simulink model "s_c_nbe_m1k"  (R2016b)
(part 3 of 198)

      settings: AttributesFormatString=Latency = %<latency>
      mask Display:
      | port_label('input', 1, 'd');
      | port_label('output', 1, 'q');
      | disp(['Z^-', num2str(latency)]);
  pipeline70 : Subsystem  AncestorBlock=casper_library_delays/pipeline  mask(pipeline){latency=2}
      mask help:
      | An explicitly laid-out delay line to avoid mapping to SRL16s
      | for use in pipelining to help achieve timing closure.
      mask init:
      | pipeline_init(gcb,'latency',latency);
      settings: AttributesFormatString=Latency = %<latency>
      mask Display:
      | port_label('input', 1, 'd');
      | port_label('output', 1, 'q');
      | disp(['Z^-', num2str(latency)]);
  pipeline71 : Subsystem  AncestorBlock=casper_library_delays/pipeline  mask(pipeline){latency=2}
      mask help:
      | An explicitly laid-out delay line to avoid mapping to SRL16s
      | for use in pipelining to help achieve timing closure.
      mask init:
      | pipeline_init(gcb,'latency',latency);
      settings: AttributesFormatString=Latency = %<latency>
      mask Display:
      | port_label('input', 1, 'd');
      | port_label('output', 1, 'q');
      | disp(['Z^-', num2str(latency)]);
  pipeline72 : Subsystem  AncestorBlock=casper_library_delays/pipeline  mask(pipeline){latency=2}
      mask help:
      | An explicitly laid-out delay line to avoid mapping to SRL16s
      | for use in pipelining to help achieve timing closure.
      mask init:
      | pipeline_init(gcb,'latency',latency);
      settings: AttributesFormatString=Latency = %<latency>
      mask Display:
      | port_label('input', 1, 'd');
      | port_label('output', 1, 'q');
      | disp(['Z^-', num2str(latency)]);
  pipeline73 : Subsystem  AncestorBlock=casper_library_delays/pipeline  mask(pipeline){latency=2}
      mask help:
      | An explicitly laid-out delay line to avoid mapping to SRL16s
      | for use in pipelining to help achieve timing closure.
      mask init:
      | pipeline_init(gcb,'latency',latency);
      settings: AttributesFormatString=Latency = %<latency>
      mask Display:
      | port_label('input', 1, 'd');
      | port_label('output', 1, 'q');
      | disp(['Z^-', num2str(latency)]);
  pipeline74 : Subsystem  AncestorBlock=casper_library_delays/pipeline  mask(pipeline){latency=2}
      mask help:
      | An explicitly laid-out delay line to avoid mapping to SRL16s
      | for use in pipelining to help achieve timing closure.
      mask init:
      | pipeline_init(gcb,'latency',latency);
      settings: AttributesFormatString=Latency = %<latency>
      mask Display:
      | port_label('input', 1, 'd');
      | port_label('output', 1, 'q');
      | disp(['Z^-', num2str(latency)]);
  pipeline75 : Subsystem  AncestorBlock=casper_library_delays/pipeline  mask(pipeline){latency=2}
      mask help:
      | An explicitly laid-out delay line to avoid mapping to SRL16s
      | for use in pipelining to help achieve timing closure.
      mask init:
      | pipeline_init(gcb,'latency',latency);
      settings: AttributesFormatString=Latency = %<latency>
      mask Display:
      | port_label('input', 1, 'd');
      | port_label('output', 1, 'q');
      | disp(['Z^-', num2str(latency)]);
  pipeline76 : Subsystem  AncestorBlock=casper_library_delays/pipeline  mask(pipeline){latency=2}
      mask help:
      | An explicitly laid-out delay line to avoid mapping to SRL16s
      | for use in pipelining to help achieve timing closure.
      mask init:
      | pipeline_init(gcb,'latency',latency);
      settings: AttributesFormatString=Latency = %<latency>
      mask Display:
      | port_label('input', 1, 'd');
      | port_label('output', 1, 'q');
      | disp(['Z^-', num2str(latency)]);
  pipeline77 : Subsystem  AncestorBlock=casper_library_delays/pipeline  mask(pipeline){latency=2}
      mask help:
      | An explicitly laid-out delay line to avoid mapping to SRL16s
      | for use in pipelining to help achieve timing closure.
      mask init:
      | pipeline_init(gcb,'latency',latency);
      settings: AttributesFormatString=Latency = %<latency>
      mask Display:
      | port_label('input', 1, 'd');
      | port_label('output', 1, 'q');
      | disp(['Z^-', num2str(latency)]);
  pipeline78 : Subsystem  AncestorBlock=casper_library_delays/pipeline  mask(pipeline){latency=2}
      mask help:
      | An explicitly laid-out delay line to avoid mapping to SRL16s
      | for use in pipelining to help achieve timing closure.
      mask init:
      | pipeline_init(gcb,'latency',latency);
      settings: AttributesFormatString=Latency = %<latency>
      mask Display:
      | port_label('input', 1, 'd');
      | port_label('output', 1, 'q');
      | disp(['Z^-', num2str(latency)]);
  pipeline79 : Subsystem  AncestorBlock=casper_library_delays/pipeline  mask(pipeline){latency=2}
      mask help:
      | An explicitly laid-out delay line to avoid mapping to SRL16s
      | for use in pipelining to help achieve timing closure.
      mask init:
      | pipeline_init(gcb,'latency',latency);
      settings: AttributesFormatString=Latency = %<latency>
      mask Display:
      | port_label('input', 1, 'd');
      | port_label('output', 1, 'q');
      | disp(['Z^-', num2str(latency)]);
  pipeline8 : Subsystem  AncestorBlock=casper_library_delays/pipeline  mask(pipeline){latency=2}
      mask help:
      | An explicitly laid-out delay line to avoid mapping to SRL16s
      | for use in pipelining to help achieve timing closure.
      mask init:
      | pipeline_init(gcb,'latency',latency);
      settings: AttributesFormatString=Latency = %<latency>
      mask Display:
      | port_label('input', 1, 'd');
      | port_label('output', 1, 'q');
      | disp(['Z^-', num2str(latency)]);
  pipeline80 : Subsystem  AncestorBlock=casper_library_delays/pipeline  mask(pipeline){latency=2}
      mask help:
      | An explicitly laid-out delay line to avoid mapping to SRL16s
      | for use in pipelining to help achieve timing closure.
      mask init:
      | pipeline_init(gcb,'latency',latency);
      settings: AttributesFormatString=Latency = %<latency>
      mask Display:
      | port_label('input', 1, 'd');
      | port_label('output', 1, 'q');
      | disp(['Z^-', num2str(latency)]);
  pipeline82 : Subsystem  AncestorBlock=casper_library_delays/pipeline  mask(pipeline){latency=2}
      mask help:
      | An explicitly laid-out delay line to avoid mapping to SRL16s
      | for use in pipelining to help achieve timing closure.
      mask init:
      | pipeline_init(gcb,'latency',latency);
      settings: AttributesFormatString=Latency = %<latency>
      mask Display:
      | port_label('input', 1, 'd');
      | port_label('output', 1, 'q');
      | disp(['Z^-', num2str(latency)]);
  pipeline83 : Subsystem  AncestorBlock=casper_library_delays/pipeline  mask(pipeline){latency=2}
      mask help:
      | An explicitly laid-out delay line to avoid mapping to SRL16s
      | for use in pipelining to help achieve timing closure.
      mask init:
      | pipeline_init(gcb,'latency',latency);
      settings: AttributesFormatString=Latency = %<latency>
      mask Display:
      | port_label('input', 1, 'd');
      | port_label('output', 1, 'q');
      | disp(['Z^-', num2str(latency)]);
  pipeline84 : Subsystem  AncestorBlock=casper_library_delays/pipeline  mask(pipeline){latency=2}
      mask help:
      | An explicitly laid-out delay line to avoid mapping to SRL16s
      | for use in pipelining to help achieve timing closure.
      mask init:
      | pipeline_init(gcb,'latency',latency);
      settings: AttributesFormatString=Latency = %<latency>
      mask Display:
      | port_label('input', 1, 'd');
      | port_label('output', 1, 'q');
      | disp(['Z^-', num2str(latency)]);
  pipeline85 : Subsystem  AncestorBlock=casper_library_delays/pipeline  mask(pipeline){latency=2}
      mask help:
      | An explicitly laid-out delay line to avoid mapping to SRL16s
      | for use in pipelining to help achieve timing closure.
      mask init:
      | pipeline_init(gcb,'latency',latency);
      settings: AttributesFormatString=Latency = %<latency>
      mask Display:
      | port_label('input', 1, 'd');
      | port_label('output', 1, 'q');
      | disp(['Z^-', num2str(latency)]);
  pipeline86 : Subsystem  AncestorBlock=casper_library_delays/pipeline  mask(pipeline){latency=2}
      mask help:
      | An explicitly laid-out delay line to avoid mapping to SRL16s
      | for use in pipelining to help achieve timing closure.
      mask init:
      | pipeline_init(gcb,'latency',latency);
      settings: AttributesFormatString=Latency = %<latency>
      mask Display:
      | port_label('input', 1, 'd');
      | port_label('output', 1, 'q');
      | disp(['Z^-', num2str(latency)]);
  pipeline87 : Subsystem  AncestorBlock=casper_library_delays/pipeline  mask(pipeline){latency=2}
      mask help:
      | An explicitly laid-out delay line to avoid mapping to SRL16s
      | for use in pipelining to help achieve timing closure.
      mask init:
      | pipeline_init(gcb,'latency',latency);
      settings: AttributesFormatString=Latency = %<latency>
      mask Display:
      | port_label('input', 1, 'd');
      | port_label('output', 1, 'q');
      | disp(['Z^-', num2str(latency)]);
  pipeline88 : Subsystem  AncestorBlock=casper_library_delays/pipeline  mask(pipeline){latency=2}
      mask help:
      | An explicitly laid-out delay line to avoid mapping to SRL16s
      | for use in pipelining to help achieve timing closure.
      mask init:
      | pipeline_init(gcb,'latency',latency);
      settings: AttributesFormatString=Latency = %<latency>
      mask Display:
      | port_label('input', 1, 'd');
      | port_label('output', 1, 'q');
      | disp(['Z^-', num2str(latency)]);
  pipeline89 : Subsystem  AncestorBlock=casper_library_delays/pipeline  mask(pipeline){latency=2}
      mask help:
      | An explicitly laid-out delay line to avoid mapping to SRL16s
      | for use in pipelining to help achieve timing closure.
      mask init:
      | pipeline_init(gcb,'latency',latency);
      settings: AttributesFormatString=Latency = %<latency>
      mask Display:
      | port_label('input', 1, 'd');
      | port_label('output', 1, 'q');
      | disp(['Z^-', num2str(latency)]);
  pipeline9 : Subsystem  AncestorBlock=casper_library_delays/pipeline  mask(pipeline){latency=2}
      mask help:
      | An explicitly laid-out delay line to avoid mapping to SRL16s
      | for use in pipelining to help achieve timing closure.
      mask init:
      | pipeline_init(gcb,'latency',latency);
      settings: AttributesFormatString=Latency = %<latency>
      mask Display:
      | port_label('input', 1, 'd');
      | port_label('output', 1, 'q');
      | disp(['Z^-', num2str(latency)]);
  pipeline90 : Subsystem  AncestorBlock=casper_library_delays/pipeline  mask(pipeline){latency=2}
      mask help:
      | An explicitly laid-out delay line to avoid mapping to SRL16s
      | for use in pipelining to help achieve timing closure.
      mask init:
      | pipeline_init(gcb,'latency',latency);
      settings: AttributesFormatString=Latency = %<latency>
      mask Display:
      | port_label('input', 1, 'd');
      | port_label('output', 1, 'q');
      | disp(['Z^-', num2str(latency)]);
  pipeline91 : Subsystem  AncestorBlock=casper_library_delays/pipeline  mask(pipeline){latency=2}
      mask help:
      | An explicitly laid-out delay line to avoid mapping to SRL16s
      | for use in pipelining to help achieve timing closure.
      mask init:
      | pipeline_init(gcb,'latency',latency);
      settings: AttributesFormatString=Latency = %<latency>
      mask Display:
      | port_label('input', 1, 'd');
      | port_label('output', 1, 'q');
      | disp(['Z^-', num2str(latency)]);
  pipeline92 : Subsystem  AncestorBlock=casper_library_delays/pipeline  mask(pipeline){latency=2}
      mask help:
      | An explicitly laid-out delay line to avoid mapping to SRL16s
      | for use in pipelining to help achieve timing closure.
      mask init:
      | pipeline_init(gcb,'latency',latency);
      settings: AttributesFormatString=Latency = %<latency>
      mask Display:
      | port_label('input', 1, 'd');
      | port_label('output', 1, 'q');
      | disp(['Z^-', num2str(latency)]);
  pipeline93 : Subsystem  AncestorBlock=casper_library_delays/pipeline  mask(pipeline){latency=2}
      mask help:
      | An explicitly laid-out delay line to avoid mapping to SRL16s
      | for use in pipelining to help achieve timing closure.
      mask init:
      | pipeline_init(gcb,'latency',latency);
      settings: AttributesFormatString=Latency = %<latency>
      mask Display:
      | port_label('input', 1, 'd');
      | port_label('output', 1, 'q');
      | disp(['Z^-', num2str(latency)]);
  pipeline94 : Subsystem  AncestorBlock=casper_library_delays/pipeline  mask(pipeline){latency=2}
      mask help:
      | An explicitly laid-out delay line to avoid mapping to SRL16s
      | for use in pipelining to help achieve timing closure.
      mask init:
      | pipeline_init(gcb,'latency',latency);
      settings: AttributesFormatString=Latency = %<latency>
      mask Display:
      | port_label('input', 1, 'd');
      | port_label('output', 1, 'q');
      | disp(['Z^-', num2str(latency)]);
  pipeline95 : Subsystem  AncestorBlock=casper_library_delays/pipeline  mask(pipeline){latency=2}
      mask help:
      | An explicitly laid-out delay line to avoid mapping to SRL16s
      | for use in pipelining to help achieve timing closure.
      mask init:
      | pipeline_init(gcb,'latency',latency);
      settings: AttributesFormatString=Latency = %<latency>
      mask Display:
      | port_label('input', 1, 'd');
      | port_label('output', 1, 'q');
      | disp(['Z^-', num2str(latency)]);
  pipeline96 : Subsystem  AncestorBlock=casper_library_delays/pipeline  mask(pipeline){latency=2}
      mask help:
      | An explicitly laid-out delay line to avoid mapping to SRL16s
      | for use in pipelining to help achieve timing closure.
      mask init:
      | pipeline_init(gcb,'latency',latency);
      settings: AttributesFormatString=Latency = %<latency>
      mask Display:
      | port_label('input', 1, 'd');
      | port_label('output', 1, 'q');
      | disp(['Z^-', num2str(latency)]);
  pipeline97 : Subsystem  AncestorBlock=casper_library_delays/pipeline  mask(pipeline){latency=2}
      mask help:
      | An explicitly laid-out delay line to avoid mapping to SRL16s
      | for use in pipelining to help achieve timing closure.
      mask init:
      | pipeline_init(gcb,'latency',latency);
      settings: AttributesFormatString=Latency = %<latency>
      mask Display:
      | port_label('input', 1, 'd');
      | port_label('output', 1, 'q');
      | disp(['Z^-', num2str(latency)]);
  pipeline98 : Subsystem  AncestorBlock=casper_library_delays/pipeline  mask(pipeline){latency=2}
      mask help:
      | An explicitly laid-out delay line to avoid mapping to SRL16s
      | for use in pipelining to help achieve timing closure.
      mask init:
      | pipeline_init(gcb,'latency',latency);
      settings: AttributesFormatString=Latency = %<latency>
      mask Display:
      | port_label('input', 1, 'd');
      | port_label('output', 1, 'q');
      | disp(['Z^-', num2str(latency)]);
  pipeline99 : Subsystem  AncestorBlock=casper_library_delays/pipeline  mask(pipeline){latency=2}
      mask help:
      | An explicitly laid-out delay line to avoid mapping to SRL16s
      | for use in pipelining to help achieve timing closure.
      mask init:
      | pipeline_init(gcb,'latency',latency);
      settings: AttributesFormatString=Latency = %<latency>
      mask Display:
      | port_label('input', 1, 'd');
      | port_label('output', 1, 'q');
      | disp(['Z^-', num2str(latency)]);
  pktlen_check : Subsystem  mask{block_len=32}
      mask prompts: block_len "Expected length"
      mask Display:
      | disp(sprintf('block_len == %i?', block_len));
      | color('green');
      | port_label('input', 1, 'pktstart')
      | port_label('input', 2, 'dv')
      | color('red');
      | port_label('output', 1, 'err')
  posedge_delay : Subsystem
  posedge_delay1 : Subsystem
  quant0 : Subsystem  mask{channel_bits=fft_stages-1, din_bit_width=18, din_bin_pt=17, coeff_bit_width=16, coeff_bin_pt=5, dout_bit_width=8, dout_bin_pt=7, overflow=Saturate, quantization=Round  (unbiased: +/- Inf), conv_latency=7, add_latency=7, mult_latency=7, bram_latency=7}
      mask prompts: channel_bits "Number channels (2^?)"; din_bit_width "Data input bit width"; din_bin_pt "Data input binary point"; coeff_bit_width "Coefficient bit width"; coeff_bin_pt "Coefficient binary point"; dout_bit_width "Data out bit width"; dout_bin_pt "Data out binary point"; overflow "Overflow behaviour"; quantization "Quantization Behaviour"; conv_latency "Conversion latency"; add_latency "Adder latency"; mult_latency "Multiplier latency"; bram_latency "BRAM latency"
      mask TypeOptions overflow: Wrap | Saturate | Error
      mask TypeOptions quantization: Truncate | Round  (unbiased: +/- Inf) | Round  (unbiased: even values)
  quant1 : Subsystem  mask{channel_bits=fft_stages-1, din_bit_width=18, din_bin_pt=17, coeff_bit_width=16, coeff_bin_pt=5, dout_bit_width=8, dout_bin_pt=7, overflow=Saturate, quantization=Round  (unbiased: +/- Inf), conv_latency=7, add_latency=7, mult_latency=7, bram_latency=7}
      mask prompts: channel_bits "Number channels (2^?)"; din_bit_width "Data input bit width"; din_bin_pt "Data input binary point"; coeff_bit_width "Coefficient bit width"; coeff_bin_pt "Coefficient binary point"; dout_bit_width "Data out bit width"; dout_bin_pt "Data out binary point"; overflow "Overflow behaviour"; quantization "Quantization Behaviour"; conv_latency "Conversion latency"; add_latency "Adder latency"; mult_latency "Multiplier latency"; bram_latency "BRAM latency"
      mask TypeOptions overflow: Wrap | Saturate | Error
      mask TypeOptions quantization: Truncate | Round  (unbiased: +/- Inf) | Round  (unbiased: even values)
  quant_pwr0 : Subsystem  Tag=xps:sw_reg  AncestorBlock=xps_library/software_register  mask(swreg){io_dir=To Processor, io_delay=0, sample_period=1, names=reg, bitwidths=32, bin_pts=31, arith_types=0, sim_port=off, show_format=off}
      mask prompts: io_dir "I/O direction"; io_delay "I/O delay"; sample_period "Sample period"; names "Bitfield names [msb...lsb]"; bitwidths "Bitfield widths"; bin_pts "Bitfield binary pts"; arith_types "Bitfield types, ufix=0, fix=1, bool=2"; sim_port "Provide sim input/output?"; show_format "Print format string?"
      mask help: A 32-bit software-accessible register. Can be divided into bitfields of varying widths and types using the fields in the block mask.
      mask init:
      | swreg_init(gcb)
      settings: AttributesFormatString=1output
      mask TypeOptions io_dir: To Processor | From Processor
      mask Callback io_dir:
      | mask_enables = get_param(gcb, 'MaskEnables');
      | mask_names = get_param(gcb, 'MaskNames');
      | if strcmp(get_param(gcb, 'io_dir'), 'To Processor'),
      |     mask_enables{ismember(mask_names, 'sample_period')} = 'off';
      | else
      |     mask_enables{ismember(mask_names, 'sample_period')} = 'on';
      | end
      | set_param(gcb, 'MaskEnables', mask_enables);
  quant_pwr1 : Subsystem  Tag=xps:sw_reg  AncestorBlock=xps_library/software_register  mask(swreg){io_dir=To Processor, io_delay=0, sample_period=1, names=reg, bitwidths=32, bin_pts=31, arith_types=0, sim_port=off, show_format=off}
      mask prompts: io_dir "I/O direction"; io_delay "I/O delay"; sample_period "Sample period"; names "Bitfield names [msb...lsb]"; bitwidths "Bitfield widths"; bin_pts "Bitfield binary pts"; arith_types "Bitfield types, ufix=0, fix=1, bool=2"; sim_port "Provide sim input/output?"; show_format "Print format string?"
      mask help: A 32-bit software-accessible register. Can be divided into bitfields of varying widths and types using the fields in the block mask.
      mask init:
      | swreg_init(gcb)
      settings: AttributesFormatString=1output
      mask TypeOptions io_dir: To Processor | From Processor
      mask Callback io_dir:
      | mask_enables = get_param(gcb, 'MaskEnables');
      | mask_names = get_param(gcb, 'MaskNames');
      | if strcmp(get_param(gcb, 'io_dir'), 'To Processor'),
      |     mask_enables{ismember(mask_names, 'sample_period')} = 'off';
      | else
      |     mask_enables{ismember(mask_names, 'sample_period')} = 'on';
      | end
      | set_param(gcb, 'MaskEnables', mask_enables);
  quant_snap_ctrl : Subsystem  Tag=xps:sw_reg  AncestorBlock=xps_library/software_register  mask(swreg){io_dir=From Processor, io_delay=0, sample_period=1, names=[single_channel channel_select], bitwidths=[1 31], bin_pts=[0 0], arith_types=[2 0], sim_port=on, show_format=on}
      mask prompts: io_dir "I/O direction"; io_delay "I/O delay"; sample_period "Sample period"; names "Bitfield names [msb...lsb]"; bitwidths "Bitfield widths"; bin_pts "Bitfield binary pts"; arith_types "Bitfield types, ufix=0, fix=1, bool=2"; sim_port "Provide sim input/output?"; show_format "Print format string?"
      mask help: A 32-bit software-accessible register. Can be divided into bitfields of varying widths and types using the fields in the block mask.
      mask init:
      | swreg_init(gcb)
      settings: AttributesFormatString=2 inputs:b,uf31.0 = 32 bits
      mask TypeOptions io_dir: To Processor | From Processor
      mask Callback io_dir:
      | mask_enables = get_param(gcb, 'MaskEnables');
      | mask_names = get_param(gcb, 'MaskNames');
      | if strcmp(get_param(gcb, 'io_dir'), 'To Processor'),
      |     mask_enables{ismember(mask_names, 'sample_period')} = 'off';
      | else
      |     mask_enables{ismember(mask_names, 'sample_period')} = 'on';
      | end
      | set_param(gcb, 'MaskEnables', mask_enables);
  quant_snap_filter0 : Subsystem
  quant_snap_filter1 : Subsystem  Commented=on
  quant_status : Subsystem  Tag=xps:sw_reg  AncestorBlock=xps_library/software register  mask(swreg){io_dir=To Processor, io_delay=0, sample_period=1, names=[pol0_or_cnt pol1_or_cnt], bitwidths=[6], bin_pts=0, arith_types=0, sim_port=off, show_format=on}
      mask prompts: io_dir "I/O direction"; io_delay "I/O delay"; sample_period "Sample period"; names "Bitfield names [msb...lsb]"; bitwidths "Bitfield widths"; bin_pts "Bitfield binary pts"; arith_types "Bitfield types, ufix=0, fix=1, bool=2"; sim_port "Provide sim input/output?"; show_format "Print format string?"
      mask help: A 32-bit software-accessible register. Can be divided into bitfields of varying widths and types using the fields in the block mask.
      mask init:
      | swreg_init(gcb)
      settings: AttributesFormatString=2 outputs:uf6.0,uf6.0 = 12 bits
      mask TypeOptions io_dir: To Processor | From Processor
      mask Callback io_dir:
      | mask_enables = get_param(gcb, 'MaskEnables');
      | mask_names = get_param(gcb, 'MaskNames');
      | if strcmp(get_param(gcb, 'io_dir'), 'To Processor'),
      |     mask_enables{ismember(mask_names, 'sample_period')} = 'off';
      | else
      |     mask_enables{ismember(mask_names, 'sample_period')} = 'on';
      | end
      | set_param(gcb, 'MaskEnables', mask_enables);
  quant_sync_cnt : Subsystem  Tag=xps:sw_reg  AncestorBlock=xps_library/Memory/software_register  mask(swreg){io_dir=To Processor, io_delay=0, init_val=0, sample_period=1, names=reg, bitwidths=8, bin_pts=0, arith_types=0, sim_port=off, show_format=on}
      mask prompts: io_dir "I/O direction"; io_delay "I/O delay"; init_val "Initial Value"; sample_period "Sample period"; names "Bitfield names [msb...lsb]"; bitwidths "Bitfield widths"; bin_pts "Bitfield binary pts"; arith_types "Bitfield types, ufix=0, fix=1, bool=2"; sim_port "Provide sim input/output?"; show_format "Print format string?"
      mask help: A 32-bit software-accessible register. Can be divided into bitfields of varying widths and types using the fields in the block mask.
      mask init:
      | swreg_init(gcb)
      settings: AttributesFormatString=1output:uf8.0 = 8 bits
      mask TypeOptions io_dir: To Processor | From Processor
      mask Callback io_dir:
      | mask_enables = get_param(gcb, 'MaskEnables');
      | mask_names = get_param(gcb, 'MaskNames');
      | if strcmp(get_param(gcb, 'io_dir'), 'To Processor'),
      |     mask_enables{ismember(mask_names, 'sample_period')} = 'off';
      | else
      |     mask_enables{ismember(mask_names, 'sample_period')} = 'on';
      | end
      | set_param(gcb, 'MaskEnables', mask_enables);
      mask DialogControl ParameterTabVar0 Prompt: Setup
  re_im_interleave : Subsystem
  reorder_status : Subsystem  Tag=xps:sw_reg  AncestorBlock=xps_library/software_register  mask(swreg){io_dir=To Processor, io_delay=0, sample_period=1, names=[timestep_err_cnt receive_err_cnt discard_cnt relock_err_cnt overflow_err_cnt dv_cnt], bitwidths=5, bin_pts=0, arith_types=0, sim_port=off, show_format=on}
      mask prompts: io_dir "I/O direction"; io_delay "I/O delay"; sample_period "Sample period"; names "Bitfield names [msb...lsb]"; bitwidths "Bitfield widths"; bin_pts "Bitfield binary pts"; arith_types "Bitfield types, ufix=0, fix=1, bool=2"; sim_port "Provide sim input/output?"; show_format "Print format string?"
      mask help: A 32-bit software-accessible register. Can be divided into bitfields of varying widths and types using the fields in the block mask.
      mask init:
      | swreg_init(gcb)
      settings: AttributesFormatString=6 outputs:uf5.0,uf5.0,uf5.0,uf5.0,uf5.0,uf5.0 = 30 bits
      mask TypeOptions io_dir: To Processor | From Processor
      mask Callback io_dir:
      | mask_enables = get_param(gcb, 'MaskEnables');
      | mask_names = get_param(gcb, 'MaskNames');
      | if strcmp(get_param(gcb, 'io_dir'), 'To Processor'),
      |     mask_enables{ismember(mask_names, 'sample_period')} = 'off';
      | else
      |     mask_enables{ismember(mask_names, 'sample_period')} = 'on';
      | end
      | set_param(gcb, 'MaskEnables', mask_enables);
  reorder_status1 : Subsystem  Tag=xps:sw_reg  AncestorBlock=xps_library/software_register  mask(swreg){io_dir=To Processor, io_delay=0, sample_period=1, names=dv_per_sec, bitwidths=32, bin_pts=0, arith_types=0, sim_port=off, show_format=on}
      mask prompts: io_dir "I/O direction"; io_delay "I/O delay"; sample_period "Sample period"; names "Bitfield names [msb...lsb]"; bitwidths "Bitfield widths"; bin_pts "Bitfield binary pts"; arith_types "Bitfield types, ufix=0, fix=1, bool=2"; sim_port "Provide sim input/output?"; show_format "Print format string?"
      mask help: A 32-bit software-accessible register. Can be divided into bitfields of varying widths and types using the fields in the block mask.
      mask init:
      | swreg_init(gcb)
      settings: AttributesFormatString=1output:uf32.0 = 32 bits
      mask TypeOptions io_dir: To Processor | From Processor
      mask Callback io_dir:
      | mask_enables = get_param(gcb, 'MaskEnables');
      | mask_names = get_param(gcb, 'MaskNames');
      | if strcmp(get_param(gcb, 'io_dir'), 'To Processor'),
      |     mask_enables{ismember(mask_names, 'sample_period')} = 'off';
      | else
      |     mask_enables{ismember(mask_names, 'sample_period')} = 'on';
      | end
      | set_param(gcb, 'MaskEnables', mask_enables);
  rx_dest_ip : Subsystem  Tag=xps:sw_reg  AncestorBlock=xps_library/software register  mask(swreg){io_dir=To Processor, io_delay=0, sample_period=1, names=reg, bitwidths=32, bin_pts=0, arith_types=0, sim_port=off, show_format=on}
      mask prompts: io_dir "I/O direction"; io_delay "I/O delay"; sample_period "Sample period"; names "Bitfield names [msb...lsb]"; bitwidths "Bitfield widths"; bin_pts "Bitfield binary pts"; arith_types "Bitfield types, ufix=0, fix=1, bool=2"; sim_port "Provide sim input/output?"; show_format "Print format string?"
      mask help: A 32-bit software-accessible register. Can be divided into bitfields of varying widths and types using the fields in the block mask.
      mask init:
      | swreg_init(gcb)
      settings: AttributesFormatString=1output:uf32.0 = 32 bits
      mask TypeOptions io_dir: To Processor | From Processor
      mask Callback io_dir:
      | mask_enables = get_param(gcb, 'MaskEnables');
      | mask_names = get_param(gcb, 'MaskNames');
      | if strcmp(get_param(gcb, 'io_dir'), 'To Processor'),
      |     mask_enables{ismember(mask_names, 'sample_period')} = 'off';
      | else
      |     mask_enables{ismember(mask_names, 'sample_period')} = 'on';
      | end
      | set_param(gcb, 'MaskEnables', mask_enables);
  snap_adc : Subsystem  Tag=casper:bitsnap  AncestorBlock=casper_library_scopes/bitfield_snapshot  mask(bitsnap){io_names=[p0_d0 p0_d1 p0_d2 p0_d3 p0_d4 p0_d5 p0_d6 p0_d7 dv sync trig trig_time], io_widths=[10 10 10 10 10 10 10 10 1 1 1 45], io_bps=[9 9 9 9 9 9 9 9 0 0 0 0], io_types=[1 1 1 1 1 1 1 1 2 2 2 0], show_format=on, snap_storage=bram, snap_dram_dimm=2, snap_dram_clock=250, snap_nsamples=8, snap_data_width=128, snap_offset=off, snap_circap=off, snap_value=off, snap_ext_arm=off, snap_ext_circ=off, snap_provide_outputs=on, snap_use_dsp48=on, snap_delay=2, extra_names=timestamp, extra_widths=32, extra_bps=0, extra_types=0}
      mask prompts: io_names "Names [msb...lsb]"; io_widths "Bitwidths [msb...lsb]"; io_bps "Binary pts [msb...lsb]"; io_types "Data types [msb...lsb], ufix=0, fix=1, bool=2"; show_format "Print format string?"; snap_storage "Storage medium"; snap_dram_dimm "DRAM dimm"; snap_dram_clock "DRAM clock rate"; snap_nsamples "Number of Samples (2^?)"; snap_data_width "Data width"; snap_offset "Start delay support"; snap_circap "Circular capture support"; snap_value "Extra value capture support"; snap_ext_arm "External arm support"; snap_ext_circ "External circular capture support"; snap_provide_outputs "Provide outputs"; snap_use_dsp48 "Use DSP48s to implement counters"; snap_delay "Pre-snapshot delay"; extra_names "Names [msb...lsb]"; extra_widths "Widths [msb...lsb]"; extra_bps "Binary pts [msb...lsb]"; extra_types "Data types [msb...lsb], ufix=0, fix=1, bool=2"
      mask help:
      | A wrapped snapshot block. Allows specification of inputs to a snapblock word so the toolflow can automatically set up the scope.
      | See documentation for snapshot for explanation of parameters.
      mask init:
      | bitsnap_init(gcb);
      settings: AttributesFormatString=|
      | snap(12):f10.9,f10.9,f10.9,f10.9,f10.9,f10.9,f10.9,f10.9,b,b,b,uf45.0 = 128 bits\n128 wide, 256 deep
      | debugID: 41370868
      mask TypeOptions snap_storage: bram | dram
      mask Callback snap_storage: bitsnap_callback();
      mask TypeOptions snap_dram_dimm: 1 | 2 | 3 | 4
      mask TypeOptions snap_dram_clock: 200 | 250 | 266 | 300 | 333
      mask TypeOptions snap_data_width: 8 | 16 | 32 | 64 | 128
      mask Callback snap_value: bitsnap_callback();
      mask Callback snap_ext_arm: bitsnap_callback();
      mask Callback snap_ext_circ: bitsnap_callback();
      mask Callback snap_provide_outputs: bitsnap_callback();
  snap_adc0 : Subsystem  Tag=casper:bitsnap  Commented=on  AncestorBlock=casper_library_scopes/bitfield_snapshot  mask(bitsnap){io_names=[p0_d0 p0_d1 p0_d2 p0_d3 p0_d4 p0_d5 p0_d6 p0_d7 dv sync], io_widths=[10 10 10 10 10 10 10 10 1 1], io_bps=[9 9 9 9 9 9 9 9 0 0], io_types=[1 1 1 1 1 1 1 1 2 2], show_format=on, snap_storage=bram, snap_dram_dimm=2, snap_dram_clock=250, snap_nsamples=10, snap_data_width=128, snap_offset=off, snap_circap=on, snap_value=on, snap_ext_arm=off, snap_ext_circ=off, snap_provide_outputs=on, snap_use_dsp48=on, snap_delay=2, extra_names=timestamp, extra_widths=32, extra_bps=0, extra_types=0}
      mask prompts: io_names "Names [msb...lsb]"; io_widths "Bitwidths [msb...lsb]"; io_bps "Binary pts [msb...lsb]"; io_types "Data types [msb...lsb], ufix=0, fix=1, bool=2"; show_format "Print format string?"; snap_storage "Storage medium"; snap_dram_dimm "DRAM dimm"; snap_dram_clock "DRAM clock rate"; snap_nsamples "Number of Samples (2^?)"; snap_data_width "Data width"; snap_offset "Start delay support"; snap_circap "Circular capture support"; snap_value "Extra value capture support"; snap_ext_arm "External arm support"; snap_ext_circ "External circular capture support"; snap_provide_outputs "Provide outputs"; snap_use_dsp48 "Use DSP48s to implement counters"; snap_delay "Pre-snapshot delay"; extra_names "Names [msb...lsb]"; extra_widths "Widths [msb...lsb]"; extra_bps "Binary pts [msb...lsb]"; extra_types "Data types [msb...lsb], ufix=0, fix=1, bool=2"
      mask help:
      | A wrapped snapshot block. Allows specification of inputs to a snapblock word so the toolflow can automatically set up the scope.
      | See documentation for snapshot for explanation of parameters.
      mask init:
      | bitsnap_init(gcb);
      settings: AttributesFormatString=|
      | snap(10):f10.9,f10.9,f10.9,f10.9,f10.9,f10.9,f10.9,f10.9,b,b = 82 bits\nextra(1):uf32.0 = 32 bits\n128 wide, 1024 deep
      | debugID: 74501914
      mask TypeOptions snap_storage: bram | dram
      mask Callback snap_storage: bitsnap_callback();
      mask TypeOptions snap_dram_dimm: 1 | 2 | 3 | 4
      mask TypeOptions snap_dram_clock: 200 | 250 | 266 | 300 | 333
      mask TypeOptions snap_data_width: 8 | 16 | 32 | 64 | 128
      mask Callback snap_value: bitsnap_callback();
      mask Callback snap_ext_arm: bitsnap_callback();
      mask Callback snap_ext_circ: bitsnap_callback();
      mask Callback snap_provide_outputs: bitsnap_callback();
  snap_adc1 : Subsystem  Tag=casper:bitsnap  Commented=on  AncestorBlock=casper_library_scopes/bitfield_snapshot  mask(bitsnap){io_names=[p1_d0 p1_d1 p1_d2 p1_d3 p1_d4 p1_d5 p1_d6 p1_d7], io_widths=10, io_bps=9, io_types=1, show_format=on, snap_storage=bram, snap_dram_dimm=2, snap_dram_clock=250, snap_nsamples=10, snap_data_width=128, snap_offset=off, snap_circap=on, snap_value=on, snap_ext_arm=off, snap_ext_circ=off, snap_provide_outputs=on, snap_use_dsp48=on, snap_delay=2, extra_names=timestamp, extra_widths=32, extra_bps=0, extra_types=0}
      mask prompts: io_names "Names [msb...lsb]"; io_widths "Bitwidths [msb...lsb]"; io_bps "Binary pts [msb...lsb]"; io_types "Data types [msb...lsb], ufix=0, fix=1, bool=2"; show_format "Print format string?"; snap_storage "Storage medium"; snap_dram_dimm "DRAM dimm"; snap_dram_clock "DRAM clock rate"; snap_nsamples "Number of Samples (2^?)"; snap_data_width "Data width"; snap_offset "Start delay support"; snap_circap "Circular capture support"; snap_value "Extra value capture support"; snap_ext_arm "External arm support"; snap_ext_circ "External circular capture support"; snap_provide_outputs "Provide outputs"; snap_use_dsp48 "Use DSP48s to implement counters"; snap_delay "Pre-snapshot delay"; extra_names "Names [msb...lsb]"; extra_widths "Widths [msb...lsb]"; extra_bps "Binary pts [msb...lsb]"; extra_types "Data types [msb...lsb], ufix=0, fix=1, bool=2"
      mask help:
      | A wrapped snapshot block. Allows specification of inputs to a snapblock word so the toolflow can automatically set up the scope.
      | See documentation for snapshot for explanation of parameters.
      mask init:
      | bitsnap_init(gcb);
      settings: AttributesFormatString=|
      | snap(8):f10.9,f10.9,f10.9,f10.9,f10.9,f10.9,f10.9,f10.9 = 80 bits\nextra(1):uf32.0 = 32 bits\n128 wide, 1024 deep
      | debugID: 74531705
      mask TypeOptions snap_storage: bram | dram
      mask Callback snap_storage: bitsnap_callback();
      mask TypeOptions snap_dram_dimm: 1 | 2 | 3 | 4
      mask TypeOptions snap_dram_clock: 200 | 250 | 266 | 300 | 333
      mask TypeOptions snap_data_width: 8 | 16 | 32 | 64 | 128
      mask Callback snap_value: bitsnap_callback();
      mask Callback snap_ext_arm: bitsnap_callback();
      mask Callback snap_ext_circ: bitsnap_callback();
      mask Callback snap_provide_outputs: bitsnap_callback();
  snap_cos : Subsystem  Tag=casper:bitsnap  AncestorBlock=casper_library_scopes/bitfield_snapshot  mask(bitsnap){io_names=[p0_d0 p0_d1 p0_d2 p0_d3 p0_d4 p0_d5 p0_d6 p0_d7 dv sync trig trig_time], io_widths=[10 10 10 10 10 10 10 10 1 1 1 44], io_bps=[9 9 9 9 9 9 9 9 0 0 0 0], io_types=[1 1 1 1 1 1 1 1 2 2 2 0], show_format=on, snap_storage=bram, snap_dram_dimm=2, snap_dram_clock=250, snap_nsamples=9, snap_data_width=128, snap_offset=off, snap_circap=off, snap_value=off, snap_ext_arm=off, snap_ext_circ=off, snap_provide_outputs=on, snap_use_dsp48=on, snap_delay=2, extra_names=timestamp, extra_widths=32, extra_bps=0, extra_types=0}
      mask prompts: io_names "Names [msb...lsb]"; io_widths "Bitwidths [msb...lsb]"; io_bps "Binary pts [msb...lsb]"; io_types "Data types [msb...lsb], ufix=0, fix=1, bool=2"; show_format "Print format string?"; snap_storage "Storage medium"; snap_dram_dimm "DRAM dimm"; snap_dram_clock "DRAM clock rate"; snap_nsamples "Number of Samples (2^?)"; snap_data_width "Data width"; snap_offset "Start delay support"; snap_circap "Circular capture support"; snap_value "Extra value capture support"; snap_ext_arm "External arm support"; snap_ext_circ "External circular capture support"; snap_provide_outputs "Provide outputs"; snap_use_dsp48 "Use DSP48s to implement counters"; snap_delay "Pre-snapshot delay"; extra_names "Names [msb...lsb]"; extra_widths "Widths [msb...lsb]"; extra_bps "Binary pts [msb...lsb]"; extra_types "Data types [msb...lsb], ufix=0, fix=1, bool=2"
      mask help:
      | A wrapped snapshot block. Allows specification of inputs to a snapblock word so the toolflow can automatically set up the scope.
      | See documentation for snapshot for explanation of parameters.
      mask init:
      | bitsnap_init(gcb);
      settings: AttributesFormatString=|
      | snap(12):f10.9,f10.9,f10.9,f10.9,f10.9,f10.9,f10.9,f10.9,b,b,b,uf44.0 = 127 bits\n128 wide, 512 deep
      | debugID: 109264557
      mask TypeOptions snap_storage: bram | dram
      mask Callback snap_storage: bitsnap_callback();
      mask TypeOptions snap_dram_dimm: 1 | 2 | 3 | 4
      mask TypeOptions snap_dram_clock: 200 | 250 | 266 | 300 | 333
      mask TypeOptions snap_data_width: 8 | 16 | 32 | 64 | 128
      mask Callback snap_value: bitsnap_callback();
      mask Callback snap_ext_arm: bitsnap_callback();
      mask Callback snap_ext_circ: bitsnap_callback();
      mask Callback snap_provide_outputs: bitsnap_callback();
  snap_dds_tg : Subsystem  Tag=casper:bitsnap  AncestorBlock=casper_library_scopes/bitfield_snapshot  mask(bitsnap){io_names=[time_slice sync dv], io_widths=[28 1 1], io_bps=[0 0 0], io_types=[0 2 2], show_format=on, snap_storage=bram, snap_dram_dimm=2, snap_dram_clock=250, snap_nsamples=9, snap_data_width=32, snap_offset=off, snap_circap=off, snap_value=off, snap_ext_arm=off, snap_ext_circ=off, snap_provide_outputs=on, snap_use_dsp48=on, snap_delay=2, extra_names=timestamp, extra_widths=32, extra_bps=0, extra_types=0}
      mask prompts: io_names "Names [msb...lsb]"; io_widths "Bitwidths [msb...lsb]"; io_bps "Binary pts [msb...lsb]"; io_types "Data types [msb...lsb], ufix=0, fix=1, bool=2"; show_format "Print format string?"; snap_storage "Storage medium"; snap_dram_dimm "DRAM dimm"; snap_dram_clock "DRAM clock rate"; snap_nsamples "Number of Samples (2^?)"; snap_data_width "Data width"; snap_offset "Start delay support"; snap_circap "Circular capture support"; snap_value "Extra value capture support"; snap_ext_arm "External arm support"; snap_ext_circ "External circular capture support"; snap_provide_outputs "Provide outputs"; snap_use_dsp48 "Use DSP48s to implement counters"; snap_delay "Pre-snapshot delay"; extra_names "Names [msb...lsb]"; extra_widths "Widths [msb...lsb]"; extra_bps "Binary pts [msb...lsb]"; extra_types "Data types [msb...lsb], ufix=0, fix=1, bool=2"
      mask help:
      | A wrapped snapshot block. Allows specification of inputs to a snapblock word so the toolflow can automatically set up the scope.
      | See documentation for snapshot for explanation of parameters.
      mask init:
      | bitsnap_init(gcb);
      settings: AttributesFormatString=|
      | snap(3):uf28.0,b,b = 30 bits\n32 wide, 512 deep
      | debugID: 44312395
      mask TypeOptions snap_storage: bram | dram
      mask Callback snap_storage: bitsnap_callback();
      mask TypeOptions snap_dram_dimm: 1 | 2 | 3 | 4
      mask TypeOptions snap_dram_clock: 200 | 250 | 266 | 300 | 333
      mask TypeOptions snap_data_width: 8 | 16 | 32 | 64 | 128
      mask Callback snap_value: bitsnap_callback();
      mask Callback snap_ext_arm: bitsnap_callback();
      mask Callback snap_ext_circ: bitsnap_callback();
      mask Callback snap_provide_outputs: bitsnap_callback();
  snap_pfbin : Subsystem  Tag=casper:bitsnap  AncestorBlock=casper_library_scopes/bitfield_snapshot  mask(bitsnap){io_names=[p0_d0 p0_d1 p0_d2 p0_d3 p0_d4 p0_d5 p0_d6 p0_d7 dv sync trig trig_time], io_widths=[10 10 10 10 10 10 10 10 1 1 1 45], io_bps=[9 9 9 9 9 9 9 9 0 0 0 0], io_types=[1 1 1 1 1 1 1 1 2 2 2 0], show_format=on, snap_storage=bram, snap_dram_dimm=2, snap_dram_clock=250, snap_nsamples=9, snap_data_width=128, snap_offset=off, snap_circap=off, snap_value=off, snap_ext_arm=off, snap_ext_circ=off, snap_provide_outputs=on, snap_use_dsp48=on, snap_delay=2, extra_names=timestamp, extra_widths=32, extra_bps=0, extra_types=0}
      mask prompts: io_names "Names [msb...lsb]"; io_widths "Bitwidths [msb...lsb]"; io_bps "Binary pts [msb...lsb]"; io_types "Data types [msb...lsb], ufix=0, fix=1, bool=2"; show_format "Print format string?"; snap_storage "Storage medium"; snap_dram_dimm "DRAM dimm"; snap_dram_clock "DRAM clock rate"; snap_nsamples "Number of Samples (2^?)"; snap_data_width "Data width"; snap_offset "Start delay support"; snap_circap "Circular capture support"; snap_value "Extra value capture support"; snap_ext_arm "External arm support"; snap_ext_circ "External circular capture support"; snap_provide_outputs "Provide outputs"; snap_use_dsp48 "Use DSP48s to implement counters"; snap_delay "Pre-snapshot delay"; extra_names "Names [msb...lsb]"; extra_widths "Widths [msb...lsb]"; extra_bps "Binary pts [msb...lsb]"; extra_types "Data types [msb...lsb], ufix=0, fix=1, bool=2"
      mask help:
      | A wrapped snapshot block. Allows specification of inputs to a snapblock word so the toolflow can automatically set up the scope.
      | See documentation for snapshot for explanation of parameters.
      mask init:
      | bitsnap_init(gcb);
      settings: AttributesFormatString=|
      | snap(12):f10.9,f10.9,f10.9,f10.9,f10.9,f10.9,f10.9,f10.9,b,b,b,uf45.0 = 128 bits\n128 wide, 512 deep
      | debugID: 53556067
      mask TypeOptions snap_storage: bram | dram
      mask Callback snap_storage: bitsnap_callback();
      mask TypeOptions snap_dram_dimm: 1 | 2 | 3 | 4
      mask TypeOptions snap_dram_clock: 200 | 250 | 266 | 300 | 333
      mask TypeOptions snap_data_width: 8 | 16 | 32 | 64 | 128
      mask Callback snap_value: bitsnap_callback();
      mask Callback snap_ext_arm: bitsnap_callback();
      mask Callback snap_ext_circ: bitsnap_callback();
      mask Callback snap_provide_outputs: bitsnap_callback();
  snap_quant0 : Subsystem  Tag=casper:bitsnap  AncestorBlock=casper_library_scopes/bitfield_snapshot  mask(bitsnap){io_names=[real0 imag0 real1 imag1 real2 imag2 real3 imag3 trig trig_time], io_widths=[8 8 8 8 8 8 8 8 1 48], io_bps=[7 7 7 7 7 7 7 7 0 0], io_types=[1 1 1 1 1 1 1 1 2 0], show_format=on, snap_storage=bram, snap_dram_dimm=2, snap_dram_clock=250, snap_nsamples=9, snap_data_width=128, snap_offset=on, snap_circap=off, snap_value=off, snap_ext_arm=off, snap_ext_circ=off, snap_provide_outputs=on, snap_use_dsp48=on, snap_delay=0, extra_names=[c d], extra_widths=[30 2], extra_bps=[0 0], extra_types=0}
      mask prompts: io_names "Names [msb...lsb]"; io_widths "Bitwidths [msb...lsb]"; io_bps "Binary pts [msb...lsb]"; io_types "Data types [msb...lsb], ufix=0, fix=1, bool=2"; show_format "Print format string?"; snap_storage "Storage medium"; snap_dram_dimm "DRAM dimm"; snap_dram_clock "DRAM clock rate"; snap_nsamples "Number of Samples (2^?)"; snap_data_width "Data width"; snap_offset "Start delay support"; snap_circap "Circular capture support"; snap_value "Extra value capture support"; snap_ext_arm "External arm support"; snap_ext_circ "External circular capture support"; snap_provide_outputs "Provide outputs"; snap_use_dsp48 "Use DSP48s to implement counters"; snap_delay "Pre-snapshot delay"; extra_names "Names [msb...lsb]"; extra_widths "Widths [msb...lsb]"; extra_bps "Binary pts [msb...lsb]"; extra_types "Data types [msb...lsb], ufix=0, fix=1, bool=2"
      mask help:
      | A wrapped snapshot block. Allows specification of inputs to a snapblock word so the toolflow can automatically set up the scope.
      | See documentation for snapshot for explanation of parameters.
      mask init:
      | bitsnap_init(gcb);
      settings: AttributesFormatString=|
      | snap(10):f8.7,f8.7,f8.7,f8.7,f8.7,f8.7,f8.7,f8.7,b,uf48.0 = 113 bits\n128 wide, 512 deep
      | debugID: 23153533
      mask TypeOptions snap_storage: bram | dram
      mask Callback snap_storage: bitsnap_callback();
      mask TypeOptions snap_dram_dimm: 1 | 2 | 3 | 4
      mask TypeOptions snap_dram_clock: 200 | 250 | 266 | 300 | 333
      mask TypeOptions snap_data_width: 8 | 16 | 32 | 64 | 128
      mask Callback snap_value: bitsnap_callback();
      mask Callback snap_ext_arm: bitsnap_callback();
      mask Callback snap_ext_circ: bitsnap_callback();
      mask Callback snap_provide_outputs: bitsnap_callback();
  snap_quant1 : Subsystem  Tag=casper:bitsnap  Commented=on  AncestorBlock=casper_library_scopes/bitfield_snapshot  mask(bitsnap){io_names=[real0 imag0 real1 imag1 real2 imag2 real3 imag3], io_widths=8, io_bps=7, io_types=1, show_format=on, snap_storage=bram, snap_dram_dimm=2, snap_dram_clock=250, snap_nsamples=10, snap_data_width=64, snap_offset=on, snap_circap=off, snap_value=off, snap_ext_arm=off, snap_ext_circ=off, snap_provide_outputs=on, snap_use_dsp48=on, snap_delay=0, extra_names=[c d], extra_widths=[30 2], extra_bps=[0 0], extra_types=0}
      mask prompts: io_names "Names [msb...lsb]"; io_widths "Bitwidths [msb...lsb]"; io_bps "Binary pts [msb...lsb]"; io_types "Data types [msb...lsb], ufix=0, fix=1, bool=2"; show_format "Print format string?"; snap_storage "Storage medium"; snap_dram_dimm "DRAM dimm"; snap_dram_clock "DRAM clock rate"; snap_nsamples "Number of Samples (2^?)"; snap_data_width "Data width"; snap_offset "Start delay support"; snap_circap "Circular capture support"; snap_value "Extra value capture support"; snap_ext_arm "External arm support"; snap_ext_circ "External circular capture support"; snap_provide_outputs "Provide outputs"; snap_use_dsp48 "Use DSP48s to implement counters"; snap_delay "Pre-snapshot delay"; extra_names "Names [msb...lsb]"; extra_widths "Widths [msb...lsb]"; extra_bps "Binary pts [msb...lsb]"; extra_types "Data types [msb...lsb], ufix=0, fix=1, bool=2"
      mask help:
      | A wrapped snapshot block. Allows specification of inputs to a snapblock word so the toolflow can automatically set up the scope.
      | See documentation for snapshot for explanation of parameters.
      mask init:
      | bitsnap_init(gcb);
      settings: AttributesFormatString=|
      | snap(8):f8.7,f8.7,f8.7,f8.7,f8.7,f8.7,f8.7,f8.7 = 64 bits\n64 wide, 1024 deep
      | debugID: 23183324
      mask TypeOptions snap_storage: bram | dram
      mask Callback snap_storage: bitsnap_callback();
      mask TypeOptions snap_dram_dimm: 1 | 2 | 3 | 4
      mask TypeOptions snap_dram_clock: 200 | 250 | 266 | 300 | 333
      mask TypeOptions snap_data_width: 8 | 16 | 32 | 64 | 128
      mask Callback snap_value: bitsnap_callback();
      mask Callback snap_ext_arm: bitsnap_callback();
      mask Callback snap_ext_circ: bitsnap_callback();
      mask Callback snap_provide_outputs: bitsnap_callback();
  snap_sync_gen : Subsystem  Tag=casper:bitsnap  AncestorBlock=casper_library_scopes/bitfield_snapshot  mask(bitsnap){io_names=[synced_delay sync_timeout pack_sync board_in_fault time synced sync_armed time_diff_err timestep_err cd_err ct_err], io_widths=[1 1 1 1 48 1 1 1 1 1 1], io_bps=0, io_types=[2 2 2 2 0 2 2 2 2 2 2], show_format=on, snap_storage=bram, snap_dram_dimm=2, snap_dram_clock=250, snap_nsamples=8, snap_data_width=64, snap_offset=off, snap_circap=on, snap_value=off, snap_ext_arm=off, snap_ext_circ=off, snap_provide_outputs=on, snap_use_dsp48=on, snap_delay=2, extra_names=timestamp, extra_widths=32, extra_bps=0, extra_types=0}
      mask prompts: io_names "Names [msb...lsb]"; io_widths "Bitwidths [msb...lsb]"; io_bps "Binary pts [msb...lsb]"; io_types "Data types [msb...lsb], ufix=0, fix=1, bool=2"; show_format "Print format string?"; snap_storage "Storage medium"; snap_dram_dimm "DRAM dimm"; snap_dram_clock "DRAM clock rate"; snap_nsamples "Number of Samples (2^?)"; snap_data_width "Data width"; snap_offset "Start delay support"; snap_circap "Circular capture support"; snap_value "Extra value capture support"; snap_ext_arm "External arm support"; snap_ext_circ "External circular capture support"; snap_provide_outputs "Provide outputs"; snap_use_dsp48 "Use DSP48s to implement counters"; snap_delay "Pre-snapshot delay"; extra_names "Names [msb...lsb]"; extra_widths "Widths [msb...lsb]"; extra_bps "Binary pts [msb...lsb]"; extra_types "Data types [msb...lsb], ufix=0, fix=1, bool=2"
      mask help:
      | A wrapped snapshot block. Allows specification of inputs to a snapblock word so the toolflow can automatically set up the scope.
      | See documentation for snapshot for explanation of parameters.
      mask init:
      | bitsnap_init(gcb);
      settings: AttributesFormatString=|
      | snap(11):b,b,b,b,uf48.0,b,b,b,b,b,b = 58 bits\n64 wide, 256 deep
      | debugID: 65383422
      mask TypeOptions snap_storage: bram | dram
      mask Callback snap_storage: bitsnap_callback();
      mask TypeOptions snap_dram_dimm: 1 | 2 | 3 | 4
      mask TypeOptions snap_dram_clock: 200 | 250 | 266 | 300 | 333
      mask TypeOptions snap_data_width: 8 | 16 | 32 | 64 | 128
      mask Callback snap_value: bitsnap_callback();
      mask Callback snap_ext_arm: bitsnap_callback();
      mask Callback snap_ext_circ: bitsnap_callback();
      mask Callback snap_provide_outputs: bitsnap_callback();
  snap_time_check : Subsystem  Tag=casper:bitsnap  Commented=on  AncestorBlock=casper_library_scopes/bitfield_snapshot  mask(bitsnap){io_names=[time80_48 pack_sync_time time_diff], io_widths=[48 48 32], io_bps=0, io_types=[0 0 1], show_format=on, snap_storage=bram, snap_dram_dimm=2, snap_dram_clock=250, snap_nsamples=8, snap_data_width=128, snap_offset=off, snap_circap=off, snap_value=off, snap_ext_arm=off, snap_ext_circ=off, snap_provide_outputs=on, snap_use_dsp48=on, snap_delay=2, extra_names=timestamp, extra_widths=32, extra_bps=0, extra_types=0}
      mask prompts: io_names "Names [msb...lsb]"; io_widths "Bitwidths [msb...lsb]"; io_bps "Binary pts [msb...lsb]"; io_types "Data types [msb...lsb], ufix=0, fix=1, bool=2"; show_format "Print format string?"; snap_storage "Storage medium"; snap_dram_dimm "DRAM dimm"; snap_dram_clock "DRAM clock rate"; snap_nsamples "Number of Samples (2^?)"; snap_data_width "Data width"; snap_offset "Start delay support"; snap_circap "Circular capture support"; snap_value "Extra value capture support"; snap_ext_arm "External arm support"; snap_ext_circ "External circular capture support"; snap_provide_outputs "Provide outputs"; snap_use_dsp48 "Use DSP48s to implement counters"; snap_delay "Pre-snapshot delay"; extra_names "Names [msb...lsb]"; extra_widths "Widths [msb...lsb]"; extra_bps "Binary pts [msb...lsb]"; extra_types "Data types [msb...lsb], ufix=0, fix=1, bool=2"
      mask help:
      | A wrapped snapshot block. Allows specification of inputs to a snapblock word so the toolflow can automatically set up the scope.
      | See documentation for snapshot for explanation of parameters.
      mask init:
      | bitsnap_init(gcb);
      settings: AttributesFormatString=|
      | snap(3):uf48.0,uf48.0,f32.0 = 128 bits\n128 wide, 256 deep
      | debugID: 49026964
      mask TypeOptions snap_storage: bram | dram
      mask Callback snap_storage: bitsnap_callback();
      mask TypeOptions snap_dram_dimm: 1 | 2 | 3 | 4
      mask TypeOptions snap_dram_clock: 200 | 250 | 266 | 300 | 333
      mask TypeOptions snap_data_width: 8 | 16 | 32 | 64 | 128
      mask Callback snap_value: bitsnap_callback();
      mask Callback snap_ext_arm: bitsnap_callback();
      mask Callback snap_ext_circ: bitsnap_callback();
      mask Callback snap_provide_outputs: bitsnap_callback();
  ss_time_trig_adc : Subsystem
  ss_time_trig_pfbin : Subsystem
  ss_time_trig_pfbin1 : Subsystem
  ss_time_trig_quant : Subsystem
  ss_trig_time_in_lsw : Subsystem  Tag=xps:sw_reg  AncestorBlock=xps_library/Memory/software_register  mask(swreg){io_dir=From Processor, io_delay=1, init_val=0, sample_period=1, names=time, bitwidths=32, bin_pts=0, arith_types=0, sim_port=on, show_format=on}
      mask prompts: io_dir "I/O direction"; io_delay "I/O delay"; init_val "Initial Value"; sample_period "Sample period"; names "Bitfield names [msb...lsb]"; bitwidths "Bitfield widths"; bin_pts "Bitfield binary pts"; arith_types "Bitfield types, ufix=0, fix=1, bool=2"; sim_port "Provide sim input/output?"; show_format "Print format string?"
      mask help: A 32-bit software-accessible register. Can be divided into bitfields of varying widths and types using the fields in the block mask.
      mask init:
      | swreg_init(gcb)
      settings: AttributesFormatString=1input:uf32.0 = 32 bits
      mask TypeOptions io_dir: To Processor | From Processor
      mask Callback io_dir:
      | mask_enables = get_param(gcb, 'MaskEnables');
      | mask_names = get_param(gcb, 'MaskNames');
      | if strcmp(get_param(gcb, 'io_dir'), 'To Processor'),
      |     mask_enables{ismember(mask_names, 'sample_period')} = 'off';
      | else
      |     mask_enables{ismember(mask_names, 'sample_period')} = 'on';
      | end
      | set_param(gcb, 'MaskEnables', mask_enables);
      mask DialogControl ParameterTabVar0 Prompt: Setup
  ss_trig_time_in_msw : Subsystem  Tag=xps:sw_reg  AncestorBlock=xps_library/Memory/software_register  mask(swreg){io_dir=From Processor, io_delay=1, init_val=0, sample_period=1, names=time, bitwidths=16, bin_pts=0, arith_types=0, sim_port=on, show_format=on}
      mask prompts: io_dir "I/O direction"; io_delay "I/O delay"; init_val "Initial Value"; sample_period "Sample period"; names "Bitfield names [msb...lsb]"; bitwidths "Bitfield widths"; bin_pts "Bitfield binary pts"; arith_types "Bitfield types, ufix=0, fix=1, bool=2"; sim_port "Provide sim input/output?"; show_format "Print format string?"
      mask help: A 32-bit software-accessible register. Can be divided into bitfields of varying widths and types using the fields in the block mask.
      mask init:
      | swreg_init(gcb)
      settings: AttributesFormatString=1input:uf16.0 = 16 bits
      mask TypeOptions io_dir: To Processor | From Processor
      mask Callback io_dir:
      | mask_enables = get_param(gcb, 'MaskEnables');
      | mask_names = get_param(gcb, 'MaskNames');
      | if strcmp(get_param(gcb, 'io_dir'), 'To Processor'),
      |     mask_enables{ismember(mask_names, 'sample_period')} = 'off';
      | else
      |     mask_enables{ismember(mask_names, 'sample_period')} = 'on';
      | end
      | set_param(gcb, 'MaskEnables', mask_enables);
      mask DialogControl ParameterTabVar0 Prompt: Setup
  sync_gen : Subsystem  mask{zerolsbs=26}
      mask prompts: zerolsbs "No. LSBs to be zero:"
  sync_mangle : Subsystem
  sync_status0 : Subsystem  Tag=xps:sw_reg  AncestorBlock=xps_library/software_register  mask(swreg){io_dir=To Processor, io_delay=0, sample_period=1, names=[synced_delay board_in_fault synced sync_armed sync_ct sync_flag sync_pack], bitwidths=[1 1 1 1 8 8 8], bin_pts=0, arith_types=[2 2 2 2 0 0 0], sim_port=off, show_format=on}
      mask prompts: io_dir "I/O direction"; io_delay "I/O delay"; sample_period "Sample period"; names "Bitfield names [msb...lsb]"; bitwidths "Bitfield widths"; bin_pts "Bitfield binary pts"; arith_types "Bitfield types, ufix=0, fix=1, bool=2"; sim_port "Provide sim input/output?"; show_format "Print format string?"
      mask help: A 32-bit software-accessible register. Can be divided into bitfields of varying widths and types using the fields in the block mask.
      mask init:
      | swreg_init(gcb)
      settings: AttributesFormatString=7 outputs:b,b,b,b,uf8.0,uf8.0,uf8.0 = 28 bits
      mask TypeOptions io_dir: To Processor | From Processor
      mask Callback io_dir:
      | mask_enables = get_param(gcb, 'MaskEnables');
      | mask_names = get_param(gcb, 'MaskNames');
      | if strcmp(get_param(gcb, 'io_dir'), 'To Processor'),
      |     mask_enables{ismember(mask_names, 'sample_period')} = 'off';
      | else
      |     mask_enables{ismember(mask_names, 'sample_period')} = 'on';
      | end
      | set_param(gcb, 'MaskEnables', mask_enables);
  sync_status1 : Subsystem  Tag=xps:sw_reg  AncestorBlock=xps_library/software register  mask(swreg){io_dir=To Processor, io_delay=0, sample_period=1, names=[timeout_resync_cnt time_diff_resync_cnt timestep_resync_cnt cd_resync_cnt ct_resync_cnt fault_clear_timeout_cnt fault_present_timeout_cnt], bitwidths=4, bin_pts=0, arith_types=0, sim_port=off, show_format=on}
      mask prompts: io_dir "I/O direction"; io_delay "I/O delay"; sample_period "Sample period"; names "Bitfield names [msb...lsb]"; bitwidths "Bitfield widths"; bin_pts "Bitfield binary pts"; arith_types "Bitfield types, ufix=0, fix=1, bool=2"; sim_port "Provide sim input/output?"; show_format "Print format string?"
      mask help: A 32-bit software-accessible register. Can be divided into bitfields of varying widths and types using the fields in the block mask.
      mask init:
      | swreg_init(gcb)
      settings: AttributesFormatString=7 outputs:uf4.0,uf4.0,uf4.0,uf4.0,uf4.0,uf4.0,uf4.0 = 28 bits
      mask TypeOptions io_dir: To Processor | From Processor
      mask Callback io_dir:
      | mask_enables = get_param(gcb, 'MaskEnables');
      | mask_names = get_param(gcb, 'MaskNames');
      | if strcmp(get_param(gcb, 'io_dir'), 'To Processor'),
      |     mask_enables{ismember(mask_names, 'sample_period')} = 'off';
      | else
      |     mask_enables{ismember(mask_names, 'sample_period')} = 'on';
      | end
      | set_param(gcb, 'MaskEnables', mask_enables);
  sync_status2 : Subsystem  Tag=xps:sw_reg  AncestorBlock=xps_library/software_register  mask(swreg){io_dir=To Processor, io_delay=0, sample_period=1, names=[sync80_cnt sync_pfb_cnt sync_fdfs_cnt sync_quant_cnt], bitwidths=8, bin_pts=0, arith_types=0, sim_port=off, show_format=on}
      mask prompts: io_dir "I/O direction"; io_delay "I/O delay"; sample_period "Sample period"; names "Bitfield names [msb...lsb]"; bitwidths "Bitfield widths"; bin_pts "Bitfield binary pts"; arith_types "Bitfield types, ufix=0, fix=1, bool=2"; sim_port "Provide sim input/output?"; show_format "Print format string?"
      mask help: A 32-bit software-accessible register. Can be divided into bitfields of varying widths and types using the fields in the block mask.
      mask init:
      | swreg_init(gcb)
      settings: AttributesFormatString=4 outputs:uf8.0,uf8.0,uf8.0,uf8.0 = 32 bits
      mask TypeOptions io_dir: To Processor | From Processor
      mask Callback io_dir:
      | mask_enables = get_param(gcb, 'MaskEnables');
      | mask_names = get_param(gcb, 'MaskNames');
      | if strcmp(get_param(gcb, 'io_dir'), 'To Processor'),
      |     mask_enables{ismember(mask_names, 'sample_period')} = 'off';
      | else
      |     mask_enables{ismember(mask_names, 'sample_period')} = 'on';
      | end
      | set_param(gcb, 'MaskEnables', mask_enables);
  sync_time_lsw : Subsystem  Tag=xps:sw_reg  AncestorBlock=xps_library/software_register  mask(swreg){io_dir=To Processor, io_delay=0, sample_period=1, names=reg, bitwidths=32, bin_pts=0, arith_types=0, sim_port=off, show_format=on}
      mask prompts: io_dir "I/O direction"; io_delay "I/O delay"; sample_period "Sample period"; names "Bitfield names [msb...lsb]"; bitwidths "Bitfield widths"; bin_pts "Bitfield binary pts"; arith_types "Bitfield types, ufix=0, fix=1, bool=2"; sim_port "Provide sim input/output?"; show_format "Print format string?"
      mask help: A 32-bit software-accessible register. Can be divided into bitfields of varying widths and types using the fields in the block mask.
      mask init:
      | swreg_init(gcb)
      settings: AttributesFormatString=1output:uf32.0 = 32 bits
      mask TypeOptions io_dir: To Processor | From Processor
      mask Callback io_dir:
      | mask_enables = get_param(gcb, 'MaskEnables');
      | mask_names = get_param(gcb, 'MaskNames');
      | if strcmp(get_param(gcb, 'io_dir'), 'To Processor'),
      |     mask_enables{ismember(mask_names, 'sample_period')} = 'off';
      | else
      |     mask_enables{ismember(mask_names, 'sample_period')} = 'on';
      | end
      | set_param(gcb, 'MaskEnables', mask_enables);
  sync_time_msw : Subsystem  Tag=xps:sw_reg  AncestorBlock=xps_library/software_register  mask(swreg){io_dir=To Processor, io_delay=0, sample_period=1, names=reg, bitwidths=16, bin_pts=0, arith_types=0, sim_port=off, show_format=on}
      mask prompts: io_dir "I/O direction"; io_delay "I/O delay"; sample_period "Sample period"; names "Bitfield names [msb...lsb]"; bitwidths "Bitfield widths"; bin_pts "Bitfield binary pts"; arith_types "Bitfield types, ufix=0, fix=1, bool=2"; sim_port "Provide sim input/output?"; show_format "Print format string?"
      mask help: A 32-bit software-accessible register. Can be divided into bitfields of varying widths and types using the fields in the block mask.
      mask init:
      | swreg_init(gcb)
      settings: AttributesFormatString=1output:uf16.0 = 16 bits
      mask TypeOptions io_dir: To Processor | From Processor
      mask Callback io_dir:
      | mask_enables = get_param(gcb, 'MaskEnables');
      | mask_names = get_param(gcb, 'MaskNames');
      | if strcmp(get_param(gcb, 'io_dir'), 'To Processor'),
      |     mask_enables{ismember(mask_names, 'sample_period')} = 'off';
      | else
      |     mask_enables{ismember(mask_names, 'sample_period')} = 'on';
      | end
      | set_param(gcb, 'MaskEnables', mask_enables);
  time_check : Subsystem  Tag=xps:sw_reg  AncestorBlock=xps_library/software register  mask(swreg){io_dir=From Processor, io_delay=0, sample_period=1, names=[max_difference], bitwidths=[32], bin_pts=[0], arith_types=[0], sim_port=off, show_format=on}
      mask prompts: io_dir "I/O direction"; io_delay "I/O delay"; sample_period "Sample period"; names "Bitfield names [msb...lsb]"; bitwidths "Bitfield widths"; bin_pts "Bitfield binary pts"; arith_types "Bitfield types, ufix=0, fix=1, bool=2"; sim_port "Provide sim input/output?"; show_format "Print format string?"
      mask help: A 32-bit software-accessible register. Can be divided into bitfields of varying widths and types using the fields in the block mask.
      mask init:
      | swreg_init(gcb)
      settings: AttributesFormatString=1input:uf32.0 = 32 bits
      mask TypeOptions io_dir: To Processor | From Processor
      mask Callback io_dir:
      | mask_enables = get_param(gcb, 'MaskEnables');
      | mask_names = get_param(gcb, 'MaskNames');
      | if strcmp(get_param(gcb, 'io_dir'), 'To Processor'),
      |     mask_enables{ismember(mask_names, 'sample_period')} = 'off';
      | else
      |     mask_enables{ismember(mask_names, 'sample_period')} = 'on';
      | end
      | set_param(gcb, 'MaskEnables', mask_enables);
  time_difference : Subsystem  Tag=xps:sw_reg  AncestorBlock=xps_library/software register  mask(swreg){io_dir=To Processor, io_delay=0, sample_period=1, names=time_difference, bitwidths=32, bin_pts=0, arith_types=1, sim_port=off, show_format=on}
      mask prompts: io_dir "I/O direction"; io_delay "I/O delay"; sample_period "Sample period"; names "Bitfield names [msb...lsb]"; bitwidths "Bitfield widths"; bin_pts "Bitfield binary pts"; arith_types "Bitfield types, ufix=0, fix=1, bool=2"; sim_port "Provide sim input/output?"; show_format "Print format string?"
      mask help: A 32-bit software-accessible register. Can be divided into bitfields of varying widths and types using the fields in the block mask.
      mask init:
      | swreg_init(gcb)
      settings: AttributesFormatString=1output:f32.0 = 32 bits
      mask TypeOptions io_dir: To Processor | From Processor
      mask Callback io_dir:
      | mask_enables = get_param(gcb, 'MaskEnables');
      | mask_names = get_param(gcb, 'MaskNames');
      | if strcmp(get_param(gcb, 'io_dir'), 'To Processor'),
      |     mask_enables{ismember(mask_names, 'sample_period')} = 'off';
      | else
      |     mask_enables{ismember(mask_names, 'sample_period')} = 'on';
      | end
      | set_param(gcb, 'MaskEnables', mask_enables);
  time_gen : Subsystem  mask{n_bits_period=fft_stages-1-2, n_bits_increment=3, n_bits_counter=48-fft_stages}
      mask prompts: n_bits_period "Period (2^?)"; n_bits_increment "Increment (2^?)"; n_bits_counter "Counter size (2^?)"
  time_gen1 : Subsystem  mask{n_bits_period=fft_stages-1-2-1+8, n_bits_increment=3, n_bits_counter=48-(fft_stages+8)}
      mask prompts: n_bits_period "Period (2^?)"; n_bits_increment "Increment (2^?)"; n_bits_counter "Counter size (2^?)"
  time_gen_cd : Subsystem  mask{n_bits_period=fft_stages-1-2, n_bits_increment=0, n_bits_counter=48-fft_stages}
      mask prompts: n_bits_period "Period (2^?)"; n_bits_increment "Increment (2^?)"; n_bits_counter "Counter size (2^?)"
  time_gen_dds : Subsystem  mask{n_bits_period=0, n_bits_increment=3, n_bits_counter=48}
      mask prompts: n_bits_period "Period (2^?)"; n_bits_increment "Increment (2^?)"; n_bits_counter "Counter size (2^?)"
  tl_cd0 : Subsystem  mask(timed_latch){n_bits_time=48-fft_stages, n_bits_quantization=fft_stages, n_bits_counters=4}
      mask prompts: n_bits_time "Number bits in time to compare"; n_bits_quantization "Time offset from lsb"; n_bits_counters "Bits in status counters"
      mask help:
      | Latches load_value when armed and current_time matches requested time.
      | current_time should be in ADC samples.
      mask init:
      | set_param([gcb,'/status'], 'bitwidths', mat2str([1, repmat(n_bits_counters, 1, 2)]));
      mask Help:
      | When armed, will latch new value when current time matches the time
      | specified. The input time should be in samples and mask settings allow
      | a portion of this to be compared to cater for quantization. Arm and latch
      | counts allow the current state, pending and missed latch events to be
      | determined.
  tl_cd0_control : Subsystem  Tag=xps:sw_reg  AncestorBlock=xps_library/software_register  mask(swreg){io_dir=From Processor, io_delay=0, sample_period=1, names=load_time_lsw, bitwidths=32, bin_pts=0, arith_types=0, sim_port=on, show_format=on}
      mask prompts: io_dir "I/O direction"; io_delay "I/O delay"; sample_period "Sample period"; names "Bitfield names [msb...lsb]"; bitwidths "Bitfield widths"; bin_pts "Bitfield binary pts"; arith_types "Bitfield types, ufix=0, fix=1, bool=2"; sim_port "Provide sim input/output?"; show_format "Print format string?"
      mask help: A 32-bit software-accessible register. Can be divided into bitfields of varying widths and types using the fields in the block mask.
      mask init:
      | swreg_init(gcb)
      settings: AttributesFormatString=1input:uf32.0 = 32 bits
      mask TypeOptions io_dir: To Processor | From Processor
      mask Callback io_dir:
      | mask_enables = get_param(gcb, 'MaskEnables');
      | mask_names = get_param(gcb, 'MaskNames');
      | if strcmp(get_param(gcb, 'io_dir'), 'To Processor'),
      |     mask_enables{ismember(mask_names, 'sample_period')} = 'off';
      | else
      |     mask_enables{ismember(mask_names, 'sample_period')} = 'on';
      | end
      | set_param(gcb, 'MaskEnables', mask_enables);
  tl_cd0_control0 : Subsystem  Tag=xps:sw_reg  AncestorBlock=xps_library/software_register  mask(swreg){io_dir=From Processor, io_delay=0, sample_period=1, names=[arm load_immediate load_time_msw], bitwidths=[1 1 16], bin_pts=[0 0 0], arith_types=[2 2 0], sim_port=on, show_format=on}
      mask prompts: io_dir "I/O direction"; io_delay "I/O delay"; sample_period "Sample period"; names "Bitfield names [msb...lsb]"; bitwidths "Bitfield widths"; bin_pts "Bitfield binary pts"; arith_types "Bitfield types, ufix=0, fix=1, bool=2"; sim_port "Provide sim input/output?"; show_format "Print format string?"
      mask help: A 32-bit software-accessible register. Can be divided into bitfields of varying widths and types using the fields in the block mask.
      mask init:
      | swreg_init(gcb)
      settings: AttributesFormatString=3 inputs:b,b,uf16.0 = 18 bits
      mask TypeOptions io_dir: To Processor | From Processor
      mask Callback io_dir:
      | mask_enables = get_param(gcb, 'MaskEnables');
      | mask_names = get_param(gcb, 'MaskNames');
      | if strcmp(get_param(gcb, 'io_dir'), 'To Processor'),
      |     mask_enables{ismember(mask_names, 'sample_period')} = 'off';
      | else
      |     mask_enables{ismember(mask_names, 'sample_period')} = 'on';
      | end
      | set_param(gcb, 'MaskEnables', mask_enables);
  tl_cd1 : Subsystem  mask(timed_latch){n_bits_time=48-fft_stages, n_bits_quantization=fft_stages, n_bits_counters=4}
      mask prompts: n_bits_time "Number bits in time to compare"; n_bits_quantization "Time offset from lsb"; n_bits_counters "Bits in status counters"
      mask help:
      | Latches load_value when armed and current_time matches requested time.
      | current_time should be in ADC samples.
      mask init:
      | set_param([gcb,'/status'], 'bitwidths', mat2str([1, repmat(n_bits_counters, 1, 2)]));
      mask Help:
      | When armed, will latch new value when current time matches the time
      | specified. The input time should be in samples and mask settings allow
      | a portion of this to be compared to cater for quantization. Arm and latch
      | counts allow the current state, pending and missed latch events to be
      | determined.
  tl_cd1_control : Subsystem  Tag=xps:sw_reg  AncestorBlock=xps_library/software_register  mask(swreg){io_dir=From Processor, io_delay=0, sample_period=1, names=load_time_lsw, bitwidths=32, bin_pts=0, arith_types=0, sim_port=on, show_format=on}
      mask prompts: io_dir "I/O direction"; io_delay "I/O delay"; sample_period "Sample period"; names "Bitfield names [msb...lsb]"; bitwidths "Bitfield widths"; bin_pts "Bitfield binary pts"; arith_types "Bitfield types, ufix=0, fix=1, bool=2"; sim_port "Provide sim input/output?"; show_format "Print format string?"
      mask help: A 32-bit software-accessible register. Can be divided into bitfields of varying widths and types using the fields in the block mask.
      mask init:
      | swreg_init(gcb)
      settings: AttributesFormatString=1input:uf32.0 = 32 bits
      mask TypeOptions io_dir: To Processor | From Processor
      mask Callback io_dir:
      | mask_enables = get_param(gcb, 'MaskEnables');
      | mask_names = get_param(gcb, 'MaskNames');
      | if strcmp(get_param(gcb, 'io_dir'), 'To Processor'),
      |     mask_enables{ismember(mask_names, 'sample_period')} = 'off';
      | else
      |     mask_enables{ismember(mask_names, 'sample_period')} = 'on';
      | end
      | set_param(gcb, 'MaskEnables', mask_enables);
  tl_cd1_control0 : Subsystem  Tag=xps:sw_reg  AncestorBlock=xps_library/software_register  mask(swreg){io_dir=From Processor, io_delay=0, sample_period=1, names=[arm load_immediate load_time_msw], bitwidths=[1 1 16], bin_pts=[0 0 0], arith_types=[2 2 0], sim_port=on, show_format=on}
      mask prompts: io_dir "I/O direction"; io_delay "I/O delay"; sample_period "Sample period"; names "Bitfield names [msb...lsb]"; bitwidths "Bitfield widths"; bin_pts "Bitfield binary pts"; arith_types "Bitfield types, ufix=0, fix=1, bool=2"; sim_port "Provide sim input/output?"; show_format "Print format string?"
      mask help: A 32-bit software-accessible register. Can be divided into bitfields of varying widths and types using the fields in the block mask.
      mask init:
      | swreg_init(gcb)
      settings: AttributesFormatString=3 inputs:b,b,uf16.0 = 18 bits
      mask TypeOptions io_dir: To Processor | From Processor
      mask Callback io_dir:
      | mask_enables = get_param(gcb, 'MaskEnables');
      | mask_names = get_param(gcb, 'MaskNames');
      | if strcmp(get_param(gcb, 'io_dir'), 'To Processor'),
      |     mask_enables{ismember(mask_names, 'sample_period')} = 'off';
      | else
      |     mask_enables{ismember(mask_names, 'sample_period')} = 'on';
      | end
      | set_param(gcb, 'MaskEnables', mask_enables);
  tl_cd_bs0 : Subsystem  mask(timed_latch){n_bits_time=48-fft_stages, n_bits_quantization=fft_stages, n_bits_counters=4}
      mask prompts: n_bits_time "Number bits in time to compare"; n_bits_quantization "Time offset from lsb"; n_bits_counters "Bits in status counters"
      mask help:
      | Latches load_value when armed and current_time matches requested time.
      | current_time should be in ADC samples.
      mask init:
      | set_param([gcb,'/status'], 'bitwidths', mat2str([1, repmat(n_bits_counters, 1, 2)]));
      mask Help:
      | When armed, will latch new value when current time matches the time
      | specified. The input time should be in samples and mask settings allow
      | a portion of this to be compared to cater for quantization. Arm and latch
      | counts allow the current state, pending and missed latch events to be
      | determined.
  tl_cd_bs1 : Subsystem  mask(timed_latch){n_bits_time=48-fft_stages, n_bits_quantization=fft_stages, n_bits_counters=4}
      mask prompts: n_bits_time "Number bits in time to compare"; n_bits_quantization "Time offset from lsb"; n_bits_counters "Bits in status counters"
      mask help:
      | Latches load_value when armed and current_time matches requested time.
      | current_time should be in ADC samples.
      mask init:
      | set_param([gcb,'/status'], 'bitwidths', mat2str([1, repmat(n_bits_counters, 1, 2)]));
      mask Help:
      | When armed, will latch new value when current time matches the time
      | specified. The input time should be in samples and mask settings allow
      | a portion of this to be compared to cater for quantization. Arm and latch
      | counts allow the current state, pending and missed latch events to be
      | determined.
  tl_fd0 : Subsystem  mask(timed_latch){n_bits_time=48-fft_stages, n_bits_quantization=fft_stages, n_bits_counters=4}
      mask prompts: n_bits_time "Number bits in time to compare"; n_bits_quantization "Time offset from lsb"; n_bits_counters "Bits in status counters"
      mask help:
      | Latches load_value when armed and current_time matches requested time.
      | current_time should be in ADC samples.
      mask init:
      | set_param([gcb,'/status'], 'bitwidths', mat2str([1, repmat(n_bits_counters, 1, 2)]));
      mask Help:
      | When armed, will latch new value when current time matches the time
      | specified. The input time should be in samples and mask settings allow
      | a portion of this to be compared to cater for quantization. Arm and latch
      | counts allow the current state, pending and missed latch events to be
      | determined.
  tl_fd1 : Subsystem  mask(timed_latch){n_bits_time=48-fft_stages, n_bits_quantization=fft_stages, n_bits_counters=4}
      mask prompts: n_bits_time "Number bits in time to compare"; n_bits_quantization "Time offset from lsb"; n_bits_counters "Bits in status counters"
      mask help:
      | Latches load_value when armed and current_time matches requested time.
      | current_time should be in ADC samples.
      mask init:
      | set_param([gcb,'/status'], 'bitwidths', mat2str([1, repmat(n_bits_counters, 1, 2)]));
      mask Help:
      | When armed, will latch new value when current time matches the time
      | specified. The input time should be in samples and mask settings allow
      | a portion of this to be compared to cater for quantization. Arm and latch
      | counts allow the current state, pending and missed latch events to be
      | determined.
  trig_level : Subsystem  Tag=xps:sw_reg  Commented=on  AncestorBlock=xps_library/software register  mask(swreg){io_dir=From Processor, io_delay=0, sample_period=1, names=level, bitwidths=10, bin_pts=9, arith_types=1, sim_port=off, show_format=on}
      mask prompts: io_dir "I/O direction"; io_delay "I/O delay"; sample_period "Sample period"; names "Bitfield names [msb...lsb]"; bitwidths "Bitfield widths"; bin_pts "Bitfield binary pts"; arith_types "Bitfield types, ufix=0, fix=1, bool=2"; sim_port "Provide sim input/output?"; show_format "Print format string?"
      mask help: A 32-bit software-accessible register. Can be divided into bitfields of varying widths and types using the fields in the block mask.
      mask init:
      | swreg_init(gcb)
      settings: AttributesFormatString=1input:f10.9 = 10 bits
      mask TypeOptions io_dir: To Processor | From Processor
      mask Callback io_dir:
      | mask_enables = get_param(gcb, 'MaskEnables');
      | mask_names = get_param(gcb, 'MaskNames');
      | if strcmp(get_param(gcb, 'io_dir'), 'To Processor'),
      |     mask_enables{ismember(mask_names, 'sample_period')} = 'off';
      | else
      |     mask_enables{ismember(mask_names, 'sample_period')} = 'on';
      | end
      | set_param(gcb, 'MaskEnables', mask_enables);
  trig_time_lsw : Subsystem  Tag=xps:sw_reg  Commented=on  AncestorBlock=xps_library/software register  mask(swreg){io_dir=From Processor, io_delay=0, sample_period=1, names=lsw, bitwidths=32, bin_pts=0, arith_types=0, sim_port=off, show_format=on}
      mask prompts: io_dir "I/O direction"; io_delay "I/O delay"; sample_period "Sample period"; names "Bitfield names [msb...lsb]"; bitwidths "Bitfield widths"; bin_pts "Bitfield binary pts"; arith_types "Bitfield types, ufix=0, fix=1, bool=2"; sim_port "Provide sim input/output?"; show_format "Print format string?"
      mask help: A 32-bit software-accessible register. Can be divided into bitfields of varying widths and types using the fields in the block mask.
      mask init:
      | swreg_init(gcb)
      settings: AttributesFormatString=1input:uf32.0 = 32 bits
      mask TypeOptions io_dir: To Processor | From Processor
      mask Callback io_dir:
      | mask_enables = get_param(gcb, 'MaskEnables');
      | mask_names = get_param(gcb, 'MaskNames');
      | if strcmp(get_param(gcb, 'io_dir'), 'To Processor'),
      |     mask_enables{ismember(mask_names, 'sample_period')} = 'off';
      | else
      |     mask_enables{ismember(mask_names, 'sample_period')} = 'on';
      | end
      | set_param(gcb, 'MaskEnables', mask_enables);
  trig_time_msw : Subsystem  Tag=xps:sw_reg  Commented=on  AncestorBlock=xps_library/software register  mask(swreg){io_dir=From Processor, io_delay=0, sample_period=1, names=msw, bitwidths=16, bin_pts=0, arith_types=0, sim_port=off, show_format=on}
      mask prompts: io_dir "I/O direction"; io_delay "I/O delay"; sample_period "Sample period"; names "Bitfield names [msb...lsb]"; bitwidths "Bitfield widths"; bin_pts "Bitfield binary pts"; arith_types "Bitfield types, ufix=0, fix=1, bool=2"; sim_port "Provide sim input/output?"; show_format "Print format string?"
      mask help: A 32-bit software-accessible register. Can be divided into bitfields of varying widths and types using the fields in the block mask.
      mask init:
      | swreg_init(gcb)
      settings: AttributesFormatString=1input:uf16.0 = 16 bits
      mask TypeOptions io_dir: To Processor | From Processor
      mask Callback io_dir:
      | mask_enables = get_param(gcb, 'MaskEnables');
      | mask_names = get_param(gcb, 'MaskNames');
      | if strcmp(get_param(gcb, 'io_dir'), 'To Processor'),
      |     mask_enables{ismember(mask_names, 'sample_period')} = 'off';
      | else
      |     mask_enables{ismember(mask_names, 'sample_period')} = 'on';
      | end
      | set_param(gcb, 'MaskEnables', mask_enables);
  ts_ss_lock : Subsystem  Tag=xps:sw_reg  AncestorBlock=xps_library/Memory/software_register  mask(swreg){io_dir=From Processor, io_delay=1, init_val=0, sample_period=1, names=en, bitwidths=1, bin_pts=0, arith_types=2, sim_port=on, show_format=on}
      mask prompts: io_dir "I/O direction"; io_delay "I/O delay"; init_val "Initial Value"; sample_period "Sample period"; names "Bitfield names [msb...lsb]"; bitwidths "Bitfield widths"; bin_pts "Bitfield binary pts"; arith_types "Bitfield types, ufix=0, fix=1, bool=2"; sim_port "Provide sim input/output?"; show_format "Print format string?"
      mask help: A 32-bit software-accessible register. Can be divided into bitfields of varying widths and types using the fields in the block mask.
      mask init:
      | swreg_init(gcb)
      settings: AttributesFormatString=1input:b = 1 bits
      mask TypeOptions io_dir: To Processor | From Processor
      mask Callback io_dir:
      | mask_enables = get_param(gcb, 'MaskEnables');
      | mask_names = get_param(gcb, 'MaskNames');
      | if strcmp(get_param(gcb, 'io_dir'), 'To Processor'),
      |     mask_enables{ismember(mask_names, 'sample_period')} = 'off';
      | else
      |     mask_enables{ismember(mask_names, 'sample_period')} = 'on';
      | end
      | set_param(gcb, 'MaskEnables', mask_enables);
      mask DialogControl ParameterTabVar0 Prompt: Setup
  ts_tvg : Subsystem
  tvg : Subsystem
  tvg_tone_levels : Subsystem  Tag=xps:sw_reg  AncestorBlock=xps_library/software_register  mask(swreg){io_dir=From Processor, io_delay=0, sample_period=1, names=[p0r p0i p1r p1i], bitwidths=8, bin_pts=7, arith_types=1, sim_port=on, show_format=on}
      mask prompts: io_dir "I/O direction"; io_delay "I/O delay"; sample_period "Sample period"; names "Bitfield names [msb...lsb]"; bitwidths "Bitfield widths"; bin_pts "Bitfield binary pts"; arith_types "Bitfield types, ufix=0, fix=1, bool=2"; sim_port "Provide sim input/output?"; show_format "Print format string?"
      mask help: A 32-bit software-accessible register. Can be divided into bitfields of varying widths and types using the fields in the block mask.
      mask init:
      | swreg_init(gcb)
      settings: AttributesFormatString=4 inputs:f8.7,f8.7,f8.7,f8.7 = 32 bits
      mask TypeOptions io_dir: To Processor | From Processor
      mask Callback io_dir:
      | mask_enables = get_param(gcb, 'MaskEnables');
      | mask_names = get_param(gcb, 'MaskNames');
      | if strcmp(get_param(gcb, 'io_dir'), 'To Processor'),
      |     mask_enables{ismember(mask_names, 'sample_period')} = 'off';
      | else
      |     mask_enables{ismember(mask_names, 'sample_period')} = 'on';
      | end
      | set_param(gcb, 'MaskEnables', mask_enables);
  tvg_tone_targets : Subsystem  Tag=xps:sw_reg  AncestorBlock=xps_library/software_register  mask(swreg){io_dir=From Processor, io_delay=0, sample_period=1, names=[p0 p1], bitwidths=fft_stages, bin_pts=0, arith_types=0, sim_port=on, show_format=on}
      mask prompts: io_dir "I/O direction"; io_delay "I/O delay"; sample_period "Sample period"; names "Bitfield names [msb...lsb]"; bitwidths "Bitfield widths"; bin_pts "Bitfield binary pts"; arith_types "Bitfield types, ufix=0, fix=1, bool=2"; sim_port "Provide sim input/output?"; show_format "Print format string?"
      mask help: A 32-bit software-accessible register. Can be divided into bitfields of varying widths and types using the fields in the block mask.
      mask init:
      | swreg_init(gcb)
      settings: AttributesFormatString=2 inputs:uf11.0,uf11.0 = 22 bits
      mask TypeOptions io_dir: To Processor | From Processor
      mask Callback io_dir:
      | mask_enables = get_param(gcb, 'MaskEnables');
      | mask_names = get_param(gcb, 'MaskNames');
      | if strcmp(get_param(gcb, 'io_dir'), 'To Processor'),
      |     mask_enables{ismember(mask_names, 'sample_period')} = 'off';
      | else
      |     mask_enables{ismember(mask_names, 'sample_period')} = 'on';
      | end
      | set_param(gcb, 'MaskEnables', mask_enables);
  tx_metadata : Subsystem  Tag=xps:sw_reg  AncestorBlock=xps_library/software register  mask(swreg){io_dir=From Processor, io_delay=0, sample_period=1, names=[porttx board_id], bitwidths=[16 8], bin_pts=0, arith_types=0, sim_port=off, show_format=on}
      mask prompts: io_dir "I/O direction"; io_delay "I/O delay"; sample_period "Sample period"; names "Bitfield names [msb...lsb]"; bitwidths "Bitfield widths"; bin_pts "Bitfield binary pts"; arith_types "Bitfield types, ufix=0, fix=1, bool=2"; sim_port "Provide sim input/output?"; show_format "Print format string?"
      mask help: A 32-bit software-accessible register. Can be divided into bitfields of varying widths and types using the fields in the block mask.
      mask init:
      | swreg_init(gcb)
      settings: AttributesFormatString=2 inputs:uf16.0,uf8.0 = 24 bits
      mask TypeOptions io_dir: To Processor | From Processor
      mask Callback io_dir:
      | mask_enables = get_param(gcb, 'MaskEnables');
      | mask_names = get_param(gcb, 'MaskNames');
      | if strcmp(get_param(gcb, 'io_dir'), 'To Processor'),
      |     mask_enables{ismember(mask_names, 'sample_period')} = 'off';
      | else
      |     mask_enables{ismember(mask_names, 'sample_period')} = 'on';
      | end
      | set_param(gcb, 'MaskEnables', mask_enables);
  unpack : Subsystem
  unpack_status : Subsystem  Tag=xps:sw_reg  AncestorBlock=xps_library/software_register  mask(swreg){io_dir=To Processor, io_delay=0, sample_period=1, names=[magic_err_cnt header_err_cnt pad_err_cnt pkt_len_err_cnt time_err_cnt], bitwidths=6, bin_pts=0, arith_types=0, sim_port=off, show_format=on}
      mask prompts: io_dir "I/O direction"; io_delay "I/O delay"; sample_period "Sample period"; names "Bitfield names [msb...lsb]"; bitwidths "Bitfield widths"; bin_pts "Bitfield binary pts"; arith_types "Bitfield types, ufix=0, fix=1, bool=2"; sim_port "Provide sim input/output?"; show_format "Print format string?"
      mask help: A 32-bit software-accessible register. Can be divided into bitfields of varying widths and types using the fields in the block mask.
      mask init:
      | swreg_init(gcb)
      settings: AttributesFormatString=5 outputs:uf6.0,uf6.0,uf6.0,uf6.0,uf6.0 = 30 bits
      mask TypeOptions io_dir: To Processor | From Processor
      mask Callback io_dir:
      | mask_enables = get_param(gcb, 'MaskEnables');
      | mask_names = get_param(gcb, 'MaskNames');
      | if strcmp(get_param(gcb, 'io_dir'), 'To Processor'),
      |     mask_enables{ismember(mask_names, 'sample_period')} = 'off';
      | else
      |     mask_enables{ismember(mask_names, 'sample_period')} = 'on';
      | end
      | set_param(gcb, 'MaskEnables', mask_enables);
  unpack_status1 : Subsystem  Tag=xps:sw_reg  AncestorBlock=xps_library/software_register  mask(swreg){io_dir=To Processor, io_delay=0, sample_period=1, names=pkt_cnt, bitwidths=32, bin_pts=0, arith_types=0, sim_port=off, show_format=on}
      mask prompts: io_dir "I/O direction"; io_delay "I/O delay"; sample_period "Sample period"; names "Bitfield names [msb...lsb]"; bitwidths "Bitfield widths"; bin_pts "Bitfield binary pts"; arith_types "Bitfield types, ufix=0, fix=1, bool=2"; sim_port "Provide sim input/output?"; show_format "Print format string?"
      mask help: A 32-bit software-accessible register. Can be divided into bitfields of varying widths and types using the fields in the block mask.
      mask init:
      | swreg_init(gcb)
      settings: AttributesFormatString=1output:uf32.0 = 32 bits
      mask TypeOptions io_dir: To Processor | From Processor
      mask Callback io_dir:
      | mask_enables = get_param(gcb, 'MaskEnables');
      | mask_names = get_param(gcb, 'MaskNames');
      | if strcmp(get_param(gcb, 'io_dir'), 'To Processor'),
      |     mask_enables{ismember(mask_names, 'sample_period')} = 'off';
      | else
      |     mask_enables{ismember(mask_names, 'sample_period')} = 'on';
      | end
      | set_param(gcb, 'MaskEnables', mask_enables);
  wb_prog_delay : Subsystem  mask{n_bits_fft=fft_stages, n_bits_cd=32}
      mask prompts: n_bits_fft "fft length (2^?)"; n_bits_cd "max coarse delay (2^?)"
  wb_prog_delay1 : Subsystem  mask{n_bits_fft=fft_stages, n_bits_cd=32}
      mask prompts: n_bits_fft "fft length (2^?)"; n_bits_cd "max coarse delay (2^?)"
  we_delay1 : Subsystem  AncestorBlock=casper_library_delays/pipeline  mask(pipeline){latency=2}
      mask help:
      | An explicitly laid-out delay line to avoid mapping to SRL16s
      | for use in pipelining to help achieve timing closure.
      mask init:
      | pipeline_init(gcb,'latency',latency);
      settings: AttributesFormatString=Latency = %<latency>
      mask Display:
      | port_label('input', 1, 'd');
      | port_label('output', 1, 'q');
      | disp(['Z^-', num2str(latency)]);
  we_delay112 : Subsystem  AncestorBlock=casper_library_delays/pipeline  mask(pipeline){latency=2}
      mask help:
      | An explicitly laid-out delay line to avoid mapping to SRL16s
      | for use in pipelining to help achieve timing closure.
      mask init:
      | pipeline_init(gcb,'latency',latency);
      settings: AttributesFormatString=Latency = %<latency>
      mask Display:
      | port_label('input', 1, 'd');
      | port_label('output', 1, 'q');
      | disp(['Z^-', num2str(latency)]);
  we_delay113 : Subsystem  AncestorBlock=casper_library_delays/pipeline  mask(pipeline){latency=2}
      mask help:
      | An explicitly laid-out delay line to avoid mapping to SRL16s
      | for use in pipelining to help achieve timing closure.
      mask init:
      | pipeline_init(gcb,'latency',latency);
      settings: AttributesFormatString=Latency = %<latency>
      mask Display:
      | port_label('input', 1, 'd');
      | port_label('output', 1, 'q');
      | disp(['Z^-', num2str(latency)]);
  we_delay114 : Subsystem  AncestorBlock=casper_library_delays/pipeline  mask(pipeline){latency=2}
      mask help:
      | An explicitly laid-out delay line to avoid mapping to SRL16s
      | for use in pipelining to help achieve timing closure.
      mask init:
      | pipeline_init(gcb,'latency',latency);
      settings: AttributesFormatString=Latency = %<latency>
      mask Display:
      | port_label('input', 1, 'd');
      | port_label('output', 1, 'q');
      | disp(['Z^-', num2str(latency)]);
  we_delay115 : Subsystem  AncestorBlock=casper_library_delays/pipeline  mask(pipeline){latency=2}
      mask help:
      | An explicitly laid-out delay line to avoid mapping to SRL16s
      | for use in pipelining to help achieve timing closure.
      mask init:
      | pipeline_init(gcb,'latency',latency);
      settings: AttributesFormatString=Latency = %<latency>
      mask Display:
      | port_label('input', 1, 'd');
      | port_label('output', 1, 'q');
      | disp(['Z^-', num2str(latency)]);
  we_delay116 : Subsystem  AncestorBlock=casper_library_delays/pipeline  mask(pipeline){latency=2}
      mask help:
      | An explicitly laid-out delay line to avoid mapping to SRL16s
      | for use in pipelining to help achieve timing closure.
      mask init:
      | pipeline_init(gcb,'latency',latency);
      settings: AttributesFormatString=Latency = %<latency>
      mask Display:
      | port_label('input', 1, 'd');
      | port_label('output', 1, 'q');
      | disp(['Z^-', num2str(latency)]);
  we_delay117 : Subsystem  AncestorBlock=casper_library_delays/pipeline  mask(pipeline){latency=2}
      mask help:
      | An explicitly laid-out delay line to avoid mapping to SRL16s
      | for use in pipelining to help achieve timing closure.
      mask init:
      | pipeline_init(gcb,'latency',latency);
      settings: AttributesFormatString=Latency = %<latency>
      mask Display:
      | port_label('input', 1, 'd');
      | port_label('output', 1, 'q');
      | disp(['Z^-', num2str(latency)]);
  we_delay124 : Subsystem  AncestorBlock=casper_library_delays/pipeline  mask(pipeline){latency=2}
      mask help:
      | An explicitly laid-out delay line to avoid mapping to SRL16s
      | for use in pipelining to help achieve timing closure.
      mask init:
      | pipeline_init(gcb,'latency',latency);
      settings: AttributesFormatString=Latency = %<latency>
      mask Display:
      | port_label('input', 1, 'd');
      | port_label('output', 1, 'q');
      | disp(['Z^-', num2str(latency)]);
  we_delay126 : Subsystem  AncestorBlock=casper_library_delays/pipeline  mask(pipeline){latency=2}
      mask help:
      | An explicitly laid-out delay line to avoid mapping to SRL16s
      | for use in pipelining to help achieve timing closure.
      mask init:
      | pipeline_init(gcb,'latency',latency);
      settings: AttributesFormatString=Latency = %<latency>
      mask Display:
      | port_label('input', 1, 'd');
      | port_label('output', 1, 'q');
      | disp(['Z^-', num2str(latency)]);
  we_delay13 : Subsystem  AncestorBlock=casper_library_delays/pipeline  mask(pipeline){latency=2}
      mask help:
      | An explicitly laid-out delay line to avoid mapping to SRL16s
      | for use in pipelining to help achieve timing closure.
      mask init:
      | pipeline_init(gcb,'latency',latency);
      settings: AttributesFormatString=Latency = %<latency>
      mask Display:
      | port_label('input', 1, 'd');
      | port_label('output', 1, 'q');
      | disp(['Z^-', num2str(latency)]);
  we_delay2 : Subsystem  AncestorBlock=casper_library_delays/pipeline  mask(pipeline){latency=2}
      mask help:
      | An explicitly laid-out delay line to avoid mapping to SRL16s
      | for use in pipelining to help achieve timing closure.
      mask init:
      | pipeline_init(gcb,'latency',latency);
      settings: AttributesFormatString=Latency = %<latency>
      mask Display:
      | port_label('input', 1, 'd');
      | port_label('output', 1, 'q');
      | disp(['Z^-', num2str(latency)]);
  we_delay29 : Subsystem  AncestorBlock=casper_library_delays/pipeline  mask(pipeline){latency=2}
      mask help:
      | An explicitly laid-out delay line to avoid mapping to SRL16s
      | for use in pipelining to help achieve timing closure.
      mask init:
      | pipeline_init(gcb,'latency',latency);
      settings: AttributesFormatString=Latency = %<latency>
      mask Display:
      | port_label('input', 1, 'd');
      | port_label('output', 1, 'q');
      | disp(['Z^-', num2str(latency)]);
  we_delay37 : Subsystem  AncestorBlock=casper_library_delays/pipeline  mask(pipeline){latency=2}
      mask help:
      | An explicitly laid-out delay line to avoid mapping to SRL16s
      | for use in pipelining to help achieve timing closure.
      mask init:
      | pipeline_init(gcb,'latency',latency);
      settings: AttributesFormatString=Latency = %<latency>
      mask Display:
      | port_label('input', 1, 'd');
      | port_label('output', 1, 'q');
      | disp(['Z^-', num2str(latency)]);
  we_delay38 : Subsystem  AncestorBlock=casper_library_delays/pipeline  mask(pipeline){latency=2}
      mask help:
      | An explicitly laid-out delay line to avoid mapping to SRL16s
      | for use in pipelining to help achieve timing closure.
      mask init:
      | pipeline_init(gcb,'latency',latency);
      settings: AttributesFormatString=Latency = %<latency>
      mask Display:
      | port_label('input', 1, 'd');
      | port_label('output', 1, 'q');
      | disp(['Z^-', num2str(latency)]);
  we_delay39 : Subsystem  AncestorBlock=casper_library_delays/pipeline  mask(pipeline){latency=2}
      mask help:
      | An explicitly laid-out delay line to avoid mapping to SRL16s
      | for use in pipelining to help achieve timing closure.
      mask init:
      | pipeline_init(gcb,'latency',latency);
      settings: AttributesFormatString=Latency = %<latency>
      mask Display:
      | port_label('input', 1, 'd');
      | port_label('output', 1, 'q');
      | disp(['Z^-', num2str(latency)]);
  we_delay41 : Subsystem  AncestorBlock=casper_library_delays/pipeline  mask(pipeline){latency=2}
      mask help:
      | An explicitly laid-out delay line to avoid mapping to SRL16s
      | for use in pipelining to help achieve timing closure.
      mask init:
      | pipeline_init(gcb,'latency',latency);
      settings: AttributesFormatString=Latency = %<latency>
      mask Display:
      | port_label('input', 1, 'd');
      | port_label('output', 1, 'q');
      | disp(['Z^-', num2str(latency)]);
  we_delay47 : Subsystem  AncestorBlock=casper_library_delays/pipeline  mask(pipeline){latency=2}
      mask help:
      | An explicitly laid-out delay line to avoid mapping to SRL16s
      | for use in pipelining to help achieve timing closure.
      mask init:
      | pipeline_init(gcb,'latency',latency);
      settings: AttributesFormatString=Latency = %<latency>
      mask Display:
      | port_label('input', 1, 'd');
      | port_label('output', 1, 'q');
      | disp(['Z^-', num2str(latency)]);
  we_delay48 : Subsystem  AncestorBlock=casper_library_delays/pipeline  mask(pipeline){latency=2}
      mask help:
      | An explicitly laid-out delay line to avoid mapping to SRL16s
      | for use in pipelining to help achieve timing closure.
      mask init:
      | pipeline_init(gcb,'latency',latency);
      settings: AttributesFormatString=Latency = %<latency>
      mask Display:
      | port_label('input', 1, 'd');
      | port_label('output', 1, 'q');
      | disp(['Z^-', num2str(latency)]);
  we_delay49 : Subsystem  AncestorBlock=casper_library_delays/pipeline  mask(pipeline){latency=2}
      mask help:
      | An explicitly laid-out delay line to avoid mapping to SRL16s
      | for use in pipelining to help achieve timing closure.
      mask init:
      | pipeline_init(gcb,'latency',latency);
      settings: AttributesFormatString=Latency = %<latency>
      mask Display:
      | port_label('input', 1, 'd');
      | port_label('output', 1, 'q');
      | disp(['Z^-', num2str(latency)]);
  we_delay50 : Subsystem  AncestorBlock=casper_library_delays/pipeline  mask(pipeline){latency=2}
      mask help:
      | An explicitly laid-out delay line to avoid mapping to SRL16s
      | for use in pipelining to help achieve timing closure.
      mask init:
      | pipeline_init(gcb,'latency',latency);
      settings: AttributesFormatString=Latency = %<latency>
      mask Display:
      | port_label('input', 1, 'd');
      | port_label('output', 1, 'q');
      | disp(['Z^-', num2str(latency)]);
  we_delay7 : Subsystem  AncestorBlock=casper_library_delays/pipeline  mask(pipeline){latency=2}
      mask help:
      | An explicitly laid-out delay line to avoid mapping to SRL16s
      | for use in pipelining to help achieve timing closure.
      mask init:
      | pipeline_init(gcb,'latency',latency);
      settings: AttributesFormatString=Latency = %<latency>
      mask Display:
      | port_label('input', 1, 'd');
      | port_label('output', 1, 'q');
      | disp(['Z^-', num2str(latency)]);
  x_setup : Subsystem  Tag=xps:sw_reg  AncestorBlock=xps_library/software_register  mask(swreg){io_dir=From Processor, io_delay=0, sample_period=1, names=[f_per_x ip_per_x num_x snap_arm pktstart_mux pack_mux pktoffset_sel], bitwidths=[15 4 9 1 1 1 1], bin_pts=[0 2 0 0 0 0 0], arith_types=[0 0 0 2 0 2 0], sim_port=off, show_format=on}
      mask prompts: io_dir "I/O direction"; io_delay "I/O delay"; sample_period "Sample period"; names "Bitfield names [msb...lsb]"; bitwidths "Bitfield widths"; bin_pts "Bitfield binary pts"; arith_types "Bitfield types, ufix=0, fix=1, bool=2"; sim_port "Provide sim input/output?"; show_format "Print format string?"
      mask help: A 32-bit software-accessible register. Can be divided into bitfields of varying widths and types using the fields in the block mask.
      mask init:
      | swreg_init(gcb)
      settings: AttributesFormatString=7 inputs:uf15.0,uf4.2,uf9.0,b,uf1.0,b,uf1.0 = 32 bits
      mask TypeOptions io_dir: To Processor | From Processor
      mask Callback io_dir:
      | mask_enables = get_param(gcb, 'MaskEnables');
      | mask_names = get_param(gcb, 'MaskNames');
      | if strcmp(get_param(gcb, 'io_dir'), 'To Processor'),
      |     mask_enables{ismember(mask_names, 'sample_period')} = 'off';
      | else
      |     mask_enables{ismember(mask_names, 'sample_period')} = 'on';
      | end
      | set_param(gcb, 'MaskEnables', mask_enables);
      mask DialogControl ParameterTabVar0 Prompt: Setup
  xsg_core_config : Subsystem  Tag=xps:xsg  AncestorBlock=xps_library/XSG_core_config  mask(xsg core config){hw_sys=SKARAB:xc7vx690t, clk_src=sys_clk, clk_rate=238, sample_period=1, synthesis_tool=XST}
      mask prompts: hw_sys "Hardware Platform"; clk_src "User IP Clock source"; clk_rate "User IP Clock Rate (MHz)"; sample_period "Sample Period"; synthesis_tool "Synthesis Tool:"
      mask help:
      | The XSG Core Config block is used to configure the System Generator design
      | for the casper_xps toolflow. Settings here are used to configure the
      | Xilinx System Generator block parameters automatically, and control toolflow
      | script  execution. It needs to be at the top level of all designs being compiled
      | with the casper_xps toolflow.
      mask init:
      | xps_xsg_conf_mask;
      mask Help: eval('xlWeb([getenv(''MLIB_ROOT''), ''\doc\html\sys_xsg_core_config\sys_xsg_core_config.html''])')
      mask TypeOptions hw_sys: ROACH:sx95t | ROACH:lx110t | ROACH2:sx475t | SNAP:xc7k160t | KC705:xc7k325t | SKARAB:xc7vx690t
      mask Callback hw_sys: xps_xsg_conf_callback
      mask TypeOptions clk_src: sys_clk | aux_clk
      mask Callback clk_src: xps_xsg_conf_callback
      mask Callback clk_rate: xps_xsg_conf_callback
      mask TypeOptions synthesis_tool: Leonardo Spectrum | Synplify | Synplify Pro | XST
      mask Display: fprintf(['MSSGE\n', hw_sys]);
  tag scope: arm_ts_ss_lock=global, arm_ts_ss_rst=global, cnt_rst=global, ct_board_hmc_offset=global, ct_chans_per_board=global, ct_chans_per_x=global, ct_chans_per_x_recip=global, ct_fake_data_error=global, ct_freq_gen_offset=global, ct_num_x_boards=global, ct_num_x_boards_recip=global, ct_num_xeng=global, ct_num_xeng_recip=global, ct_rst_err_latch=global, ct_tag_insert_sel=global, ct_tvg_en2=global, ct_tvg_en=global, ct_x_per_board=global, ct_x_per_board_recip=global, force_gbe_txen=global, local_time_capture=global, local_time_src=global, obuf_read_gap=global, pfb_bypass=global, pktoffset_sel=global, pktstart_sel=global, reo_time_change=global, snap_reord_mux_we_sel=global, snap_stop_mux_sel=global, ss_trig_time_in=global, sys_rst=global, tg_dds_time_out=global, tg_rd_time_out=global, time80_48=global, ts_ss_lock=global, ts_tvg_en=global, tvgtone_level0=global, tvgtone_level1=global, tvgtone_p0=global, tvgtone_p1=global, up_timestep_error=global
  wires:
  Counter2/1 -> pipeline29/1(d)
  Constant26/1 -> eq1/2(data_in)
  Constant11/1 -> eq1/3(we)
  Delay53/1 -> quant1/1(sync_in)
  Delay34/1 -> quant1/2(din)
  eq1/1(data_out) -> quant1/4(coeffs)
  Delay50/1 -> quant1/3(en)
  Counter4/1 -> pipeline27/1(d)
  Constant24/1 -> eq0/2(data_in)
  Constant25/1 -> eq0/3(we)
  Delay51/1 -> quant0/1(sync_in)
  Delay2/1 -> quant0/2(din)
  Delay52/1 -> quant0/3(en)
  eq0/1(data_out) -> quant0/4(coeffs)
  quant0/1(sync_out) -> [q_sync]
  quant0/2(dout) -> [q_d64_0]
  quant0/3(dvalid) -> [q_dv]
  quant0/4(of) -> [q_of0]
  quant1/2(dout) -> [q_d64_1]
  quant1/1(sync_out) -> Terminator19/1
  quant1/3(dvalid) -> Terminator21/1
  quant1/4(of) -> [q_of1]
  pipeline27/1(q) -> eq0/1(addr)
  pipeline29/1(q) -> eq1/1(addr)
  [fdfs_sync] -> Delay51/1, pipeline42/1(d)
  [fdfs_d144_0] -> Delay2/1
  [fdfs_dv] -> Delay52/1, pipeline41/1(d)
  pipeline41/1(q) -> Counter4/2
  pipeline42/1(q) -> Counter4/1
  pipeline45/1(q) -> Counter2/2
  [fdfs_sync] -> Delay53/1, pipeline48/1(d)
  [fdfs_d144_1] -> Delay34/1
  [fdfs_dv] -> Delay50/1, pipeline45/1(d)
  pipeline48/1(q) -> Counter2/1
  [cd_bypass] -> Mux4/1
  [cd_bypass] -> Mux2/1
  Mux4/1 -> [pfbin_sync]
  Mux2/1 -> [pfbin_dv]
  [cd_bypass] -> Mux3/1
  Mux3/1 -> [pfbin_d0]
  [cd_bypass] -> Mux5/1
  Mux5/1 -> [pfbin_d1]
  tl_cd0_control0/3(in_load_time_msw) -> Concat6/1
  tl_cd0_control/1(in_load_time_lsw) -> Concat6/2
  Constant42/1 -> tl_cd0_control/1(sim_1)
  Constant40/1 -> tl_cd0_control0/3(sim_3)
  Constant41/1 -> tl_cd0_control0/2(sim_2)
  Constant43/1 -> Delay12/1
  Delay12/1 -> tl_cd0_control0/1(sim_1)
  Concat6/1 -> pipeline136/1(d)
  tl_cd0_control0/2(in_load_immediate) -> pipeline135/1(d)
  tl_cd0_control0/1(in_arm) -> pipeline134/1(d)
  tl_cd1_control0/3(in_load_time_msw) -> Concat8/1
  tl_cd1_control/1(in_load_time_lsw) -> Concat8/2
  Constant47/1 -> tl_cd1_control/1(sim_1)
  Constant45/1 -> tl_cd1_control0/3(sim_3)
  Constant46/1 -> tl_cd1_control0/2(sim_2)
  Constant48/1 -> Delay13/1
  Delay13/1 -> tl_cd1_control0/1(sim_1)
  Concat8/1 -> pipeline143/1(d)
  tl_cd1_control0/2(in_load_immediate) -> pipeline138/1(d)
  tl_cd1_control0/1(in_arm) -> pipeline137/1(d)
  [delay_sync] -> Mux4/2
  [sync80] -> Mux4/3
  [delay_d0] -> Mux3/2
  [d80_adc0] -> Mux3/3
  [delay_d1] -> Mux5/2
  [d80_adc1] -> Mux5/3
  [valid80] -> Mux2/3
  [delay_dv] -> Mux2/2
  pipeline134/1(q) -> [tl_cd0_arm]
  pipeline135/1(q) -> [tl_cd0_load_immediate]
  pipeline136/1(q) -> [tl_cd0_load_time]
  pipeline138/1(q) -> [tl_cd1_load_immediate]
  pipeline137/1(q) -> [tl_cd1_arm]
  pipeline143/1(q) -> [tl_cd1_load_time]
  [q_sync] -> generate_pkt_sync1/1(sync)
  Concat4/1 -> generate_pkt_sync1/3(data)
  [q_d64_0] -> Concat4/1
  [q_d64_1] -> Concat4/2
  bus_expand5/1(msb_out2) -> quant_snap_filter0/3(data_in)
  [q_dv] -> generate_pkt_sync1/2(valid)
  generate_pkt_sync1/3(out_data) -> pipeline65/1(d)
  generate_pkt_sync1/2(out_valid) -> pipeline79/1(d), pipeline58/1(d)
  generate_pkt_sync1/4(packet_sync) -> pipeline80/1(d), pipeline64/1(d)
  pipeline65/1(q) -> bus_expand5/1(bus_in)
  bus_expand3/1(msb_out8) -> pipeline220/1(d)
  bus_expand3/2(out7) -> pipeline221/1(d)
  bus_expand3/3(out6) -> pipeline218/1(d)
  bus_expand3/4(out5) -> pipeline219/1(d)
  bus_expand3/5(out4) -> pipeline215/1(d)
  bus_expand3/6(out3) -> pipeline217/1(d)
  bus_expand3/7(out2) -> pipeline201/1(d)
  bus_expand3/8(lsb_out1) -> pipeline214/1(d)
  bus_expand4/1(msb_out8) -> snap_quant1/1(in_real0)
  bus_expand4/2(out7) -> snap_quant1/2(in_imag0)
  bus_expand4/3(out6) -> snap_quant1/3(in_real1)
  bus_expand4/4(out5) -> snap_quant1/4(in_imag1)
  bus_expand4/5(out4) -> snap_quant1/5(in_real2)
  bus_expand4/6(out3) -> snap_quant1/6(in_imag2)
  bus_expand4/7(out2) -> snap_quant1/7(in_real3)
  bus_expand4/8(lsb_out1) -> snap_quant1/8(in_imag3)
  quant_snap_filter0/2(data_out) -> bus_expand3/1(bus_in)
  quant_snap_filter0/1(data_valid_out) -> pipeline222/1(d)
  quant_snap_filter1/2(data_out) -> bus_expand4/1(bus_in)
  bus_expand5/2(lsb_out1) -> quant_snap_filter1/3(data_in)
  quant_snap_filter1/3(packet_sync_out) -> snap_quant1/10(trig)
  quant_snap_filter1/1(data_valid_out) -> snap_quant1/9(we)
  generate_pkt_sync1/1(out_sync) -> [generate_pkt_sync_out]
  [generate_pkt_sync_out] -> quant_snap_filter0/1(sync_in)
  From235/1 -> quant_snap_filter1/1(sync_in)
  pipeline79/1(q) -> [gp_dv0]
  [gp_dv0] -> quant_snap_filter0/2(data_valid_in)
  pipeline80/1(q) -> [gp_pktsync0]
  [gp_pktsync0] -> quant_snap_filter0/4(packet_sync_in)
  pipeline58/1(q) -> [gp_dv1]
  pipeline64/1(q) -> [gp_pktsync1]
  From233/1 -> quant_snap_filter1/2(data_valid_in)
  From215/1 -> quant_snap_filter1/4(packet_sync_in)
  [quant_snap_single_channel] -> quant_snap_filter0/5(single_channel_enable)
  [quant_snap_channel_select] -> quant_snap_filter0/6(channel_select)
  From220/1 -> quant_snap_filter1/5(single_channel_enable)
  From222/1 -> quant_snap_filter1/6(channel_select)
  Slice3/1 -> [quant_snap_channel_select]
  [hmc_sync_p0] -> pipeline139/1(d)
  [sys_rst] -> pipeline133/1(d)
  [sync80] -> pipeline129/1(d)
  [sys_rst] -> pipeline123/1(d)
  [tg_dds_data_p0] -> complexify/1(In1)
  [tg_dds_data_p1] -> complexify1/1(In1)
  [tg_dds_sync] -> Delay109/1
  [tg_dds_dvalid] -> Delay108/1
  Delay111/1 -> Delay129/1
  Delay113/1 -> Delay132/1
  DDC/1(ddc_sync) -> [ddc_sync]
  DDC/2(ddc_pol0) -> [ddc_pol0]
  DDC/3(ddc_pol1) -> [ddc_pol1]
  DDC/4(ddc_dv) -> [ddc_dvalid]
  Gateway Out65/1 -> To Workspace69/1
  [ddc_dvalid] -> Gateway Out65/1
  Gateway Out4/1 -> To Workspace1/1
  [ddc_pol1] -> Gateway Out4/1
  Gateway Out2/1 -> To Workspace2/1
  [ddc_pol0] -> Gateway Out2/1
  [ddc_sync] -> Gateway Out1/1
  Gateway Out1/1 -> To Workspace3/1
  [ddc_sync] -> pipeline145/1(d)
  [cnt_rst] -> pipeline146/1(d)
  [ddc_dvalid] -> pipeline144/1(d)
  [cnt_rst] -> pipeline142/1(d)
  [ddc_sync_in] -> DDC/1(sync)
  [ddc_pol1_in] -> DDC/5(pol1_data)
  Mux6/1 -> DDC/6(osc1), DDC/4(osc0)
  [osc_cmplx] -> Mux6/2
  [ddc_pol0_in] -> Mux6/3
  Constant31/1 -> osc_sel/1(sim_1)
  osc_sel/1(in_sel) -> Mux6/1
  [ddc_dv_in] -> DDC/2(dvalid)
  [ddc_pol0_in] -> DDC/3(pol0_data)
  [ddc_sync_in] -> pipeline141/1(d)
  [cnt_rst] -> pipeline140/1(d)
  [clr_status] -> Subsystem5/1(rst)
  Slice22/1 -> Subsystem5/2(in0)
  [pfb_of] -> Slice22/1, Slice21/1
  Slice21/1 -> Subsystem5/3(in1)
  [pfb_sync] -> Subsystem5/4(in2)
  [pfb_sync] -> pipeline153/1(d)
  [cnt_rst] -> pipeline154/1(d)
  [pfb_dv] -> pipeline151/1(d)
  [cnt_rst] -> pipeline152/1(d)
  Subsystem5/3(out2) -> pfb_status/3(out_sync_cnt)
  Subsystem5/2(out1) -> pfb_status/2(out_pol1_or_err_cnt)
  Subsystem5/1(out0) -> pfb_status/1(out_pol0_or_err_cnt)
  nb_pfb/2(dv_out) -> Delay128/1
  [ddc_sync] -> nb_pfb/1(sync)
  nb_pfb/1(sync_out) -> Delay127/1
  [clr_status] -> Subsystem15/1(rst)
  Subsystem15/1(out0) -> quant_status/1(out_pol0_or_cnt)
  Relational/1 -> Subsystem15/2(in0)
  Constant59/1 -> Relational/2
  [q_of0] -> Relational/1
  Relational3/1 -> Subsystem15/3(in1)
  [q_of1] -> Relational3/1
  Constant58/1 -> Relational3/2
  Subsystem15/2(out1) -> quant_status/2(out_pol1_or_cnt)
  tl_fd0/1(value) -> phase_compensation0/4(delay_value), Gateway Out45/1
  [clr_status] -> tl_fd1/1(rst), tl_fd0/1(rst)
  phase_compensation1/1(sync_out) -> Terminator24/1
  phase_compensation1/2(dout) -> [fdfs_d144_1]
  phase_compensation1/3(dvalid) -> Terminator25/1
  [ld_val0] -> tl_fd0/3(load_value)
  [ld_val1] -> tl_fd1/3(load_value)
  bus_expand16/1(msb_out2) -> tl_fd0/5(din)
  bus_expand16/2(lsb_out1) -> tl_fd1/5(din)
  Constant66/1 -> Concat2/2
  Concat2/1 -> tl_fd1/2(current_time), tl_fd0/2(current_time), [pfb_time]
  tl_fd0/7(misco) -> Terminator3/1
  tl_fd0/6(time) -> [fdfs_time]
  tl_fd1/6(time) -> Terminator17/1
  tl_fd1/7(misco) -> Terminator20/1
  Constant18/1 -> tl_fd0/7(misci)
  Constant29/1 -> tl_fd1/7(misci)
  time_gen/1(rd_sync_out) -> [tg_pfb_sync], tl_fd1/4(sync_in), tl_fd0/4(sync_in)
  time_gen/2(rd_dvalid) -> [tg_pfb_dv], tl_fd1/6(en), tl_fd0/6(en)
  time_gen/3(rd_val_out) -> Concat2/1
  time_gen/4(rd_misc_out) -> bus_expand16/1(bus_in)
  [sync80] -> pipeline207/1(d)
  [valid80] -> pipeline208/1(d)
  [pfb_sync] -> pipeline210/1(d)
  [pfb_dv] -> pipeline212/1(d)
  [pfb_d144_1] -> pipeline231/1(d)
  [pfb_d144_0] -> pipeline228/1(d)
  Concat1/1 -> time_gen/6(rd_misc_in)
  [tl_cd0_arm] -> tl_fd0/8(arm)
  [tl_cd0_load_immediate] -> tl_fd0/9(load_immediate)
  [tl_cd1_arm] -> tl_fd1/8(arm)
  [tl_cd1_load_immediate] -> tl_fd1/9(load_immediate)
  pipeline207/1(q) -> time_gen/1(wr_sync_in)
  pipeline208/1(q) -> time_gen/2(wr_en)
  pipeline210/1(q) -> time_gen/4(rd_sync_in)
  pipeline212/1(q) -> time_gen/5(rd_en)
  pipeline228/1(q) -> Concat1/1
  pipeline231/1(q) -> Concat1/2
  Gateway Out45/1 -> To Workspace45/1
  Gateway Out46/1 -> To Workspace46/1
  [ld_val0] -> Gateway Out46/1
  tl_fd0/3(sync_out) -> phase_compensation0/1(sync_in)
  tl_fd0/4(dout) -> phase_compensation0/2(din)
  tl_fd0/5(dvalid) -> phase_compensation0/3(en)
  tl_fd0/2(enable) -> phase_compensation0/5(load_value)
  phase_compensation0/1(sync_out) -> [fdfs_sync]
  phase_compensation0/2(dout) -> [fdfs_d144_0]
  phase_compensation0/3(dvalid) -> [fdfs_dv]
  [dds_fft_phase_offset] -> phase_compensation1/6(fft_idx_offset), phase_compensation0/6(fft_idx_offset)
  [q_sync] -> pipeline158/1(d)
  [cnt_rst] -> pipeline83/1(d)
  Counter14/1 -> pipeline178/1(d)
  Constant4/1 -> gbe0/8(rx_overrun_ack)
  Constant19/1 -> gbe0/7(rx_ack)
  [gbe_rst] -> pipeline99/1(d)
  sync_gen/2(dout) -> bus_expand6/1(bus_in)
  sync_gen/3(dvalid) -> impulse_gen1/6(en), impulse_gen0/6(en)
  Slice12/1 -> [time80]
  impulse_gen0/3(dvalid) -> [valid80]
  impulse_gen0/1(sync_out) -> [sync80]
  impulse_gen0/2(dout) -> [d80_adc0]
  impulse_gen0/4(misco) -> [time80_48], Slice12/1
  [tvg_adc0_en] -> impulse_gen0/1(tvg_en)
  impulse_gen1/1(sync_out) -> Terminator6/1
  impulse_gen1/2(dout) -> [d80_adc1]
  impulse_gen1/3(dvalid) -> Terminator8/1
  impulse_gen1/4(misco) -> [dig_flags]
  [tvg_adc1_en] -> impulse_gen1/1(tvg_en)
  impulse0/1(in_offset) -> Slice7/1
  impulse0/2(in_amplitude) -> impulse_gen0/3(impulse_amplitude)
  impulse1/1(in_offset) -> Slice8/1
  impulse1/2(in_amplitude) -> impulse_gen1/3(impulse_amplitude)
  sync_gen/1(sync) -> impulse_gen0/4(sync_in), impulse_gen1/4(sync_in)
  bus_expand6/1(msb_out2) -> impulse_gen0/5(din)
  bus_expand6/2(lsb_out1) -> impulse_gen1/5(din)
  sync_gen/5(misco) -> impulse_gen1/7(misci)
  sync_gen/4(time_out) -> impulse_gen0/7(misci)
  [unpack_timestamp] -> sync_gen/1(time_in)
  [sys_relock] -> sync_gen/5(relock)
  [unpack_dv] -> sync_gen/2(en)
  [unpack_d160] -> sync_gen/3(din)
  Slice7/1 -> impulse_gen0/2(impulse_offset)
  Slice8/1 -> impulse_gen1/2(impulse_offset)
  [gbe_cnt_rst] -> pipeline31/1(d)
  pipeline31/1(q) -> gbe0/9(debug_rst)
  gbe0/13(rx_dest_ip) -> pipeline115/1(d)
  gbe0/14(rx_dest_port) -> pipeline116/1(d)
  [rx_dest_ip] -> pipeline/1(d)
  pipeline/1(q) -> rx_dest_ip/1(out_reg)
  gbe0/1(led_up) -> pipeline100/1(d)
  [forty_gbe_led_up] -> pipeline19/1(d)
  gbe0/2(led_rx) -> pipeline101/1(d)
  [forty_gbe_led_rx] -> pipeline20/1(d)
  gbe0/3(led_tx) -> pipeline102/1(d)
  [forty_gbe_led_tx] -> pipeline51/1(d)
  gbe0/4(tx_afull) -> pipeline103/1(d)
  gbe0/5(tx_overflow) -> pipeline104/1(d)
  gbe0/12(rx_overrun) -> pipeline114/1(d)
  pipeline19/1(q) -> gbe_status/1(out_led_up)
  pipeline20/1(q) -> gbe_status/2(out_led_rx)
  pipeline51/1(q) -> gbe_status/3(out_led_tx)
  gbe0/8(rx_source_ip) -> pipeline110/1(d)
  gbe0/9(rx_source_port) -> pipeline111/1(d)
  gbe0/6(rx_data) -> pipeline108/1(d)
  gbe0/10(rx_end_of_frame) -> pipeline112/1(d)
  gbe0/11(rx_bad_frame) -> pipeline113/1(d)
  [s256_d] -> pipeline98/1(d)
  [s256_ip] -> pipeline97/1(d)
  [s256_port] -> pipeline96/1(d)
  Logical3/1 -> gbe0/6(tx_end_of_frame)
  [s256_v] -> Logical1/2
  [s256_eof] -> Logical3/2
  Delay1/1 -> Logical1/1, Logical3/1
  [s256_eof] -> Delay1/2
  pipeline96/1(q) -> gbe0/5(tx_dest_port)
  pipeline97/1(q) -> gbe0/4(tx_dest_ip)
  pipeline98/1(q) -> gbe0/2(tx_data)
  pipeline99/1(q) -> gbe0/1(rst)
  Logical5/1 -> Delay1/1
  pipeline100/1(q) -> [forty_gbe_led_up]
  pipeline101/1(q) -> [forty_gbe_led_rx]
  pipeline102/1(q) -> [forty_gbe_led_tx]
  pipeline103/1(q) -> [forty_gbe_tx_full]
  pipeline104/1(q) -> [forty_gbe_tx_of]
  pipeline108/1(q) -> [forty_gbe_rx_data]
  pipeline110/1(q) -> [forty_gbe_rx_src_ip]
  pipeline111/1(q) -> [forty_gbe_rx_src_port]
  pipeline112/1(q) -> [forty_gbe_rx_eof]
  pipeline113/1(q) -> [forty_gbe_rx_bad]
  pipeline114/1(q) -> [forty_gbe_rx_overrun]
  pipeline115/1(q) -> [rx_dest_ip]
  pipeline116/1(q) -> [rx_dest_port]
  [forty_gbe_rx_data] -> unpack/1(d256)
  [forty_gbe_rx_valid] -> unpack/2(dv256)
  [forty_gbe_rx_eof] -> unpack/3(eof256)
  Constant1/1 -> sync_gen/4(misci)
  Logical1/1 -> gbe0/3(tx_valid)
  Subsystem7/1(per_sec) -> reorder_status1/1(out_dv_per_sec)
  [upg_reo_time] -> Subsystem1/3(time)
  [upg_reo_recv] -> Subsystem1/4(recv)
  [upg_reo_dv] -> Subsystem7/1(dv), Subsystem1/2(dv)
  [cnt_rst] -> Subsystem1/1(rst)
  Subsystem1/7(time_change) -> [reo_time_change]
  Logical6/1 -> Subsystem1/7(overflow_err)
  [upg_of80_p1] -> Logical6/2
  [upg_of80_p0] -> Logical6/1
  Subsystem1/8(timestep_err) -> [up_timestep_error]
  [upg_reo_disc] -> Subsystem1/5(discard_err)
  [upg_reo_relock] -> Subsystem1/6(relock_err)
  Subsystem1/1(timestep_err_cnt) -> reorder_status/1(out_timestep_err_cnt)
  Subsystem1/2(recv_err_cnt) -> reorder_status/2(out_receive_err_cnt)
  Subsystem1/3(discard_err_cnt) -> reorder_status/3(out_discard_cnt)
  Subsystem1/4(relock_err_cnt) -> reorder_status/4(out_relock_err_cnt)
  Subsystem1/5(overflow_err_cnt) -> reorder_status/5(out_overflow_err_cnt)
  Subsystem1/6(dv_cnt) -> reorder_status/6(out_dv_cnt)
  gbe0/7(rx_valid) -> pipeline62/1(d)
  pipeline62/1(q) -> [forty_gbe_rx_valid]
  [gbe_txen] -> Logical5/2
  [force_gbe_txen] -> Logical7/2
  Logical7/1 -> Logical5/1
  [upg_sperr_magic] -> Subsystem33/2(in0)
  [upg_sperr_len] -> Subsystem33/5(in3)
  [upg_sperr_hdr] -> Subsystem33/3(in1)
  [upg_sperr_pad] -> Subsystem33/4(in2)
  Subsystem33/5(out4) -> unpack_status/5(out_time_err_cnt)
  [upg_sperr_time] -> Subsystem33/6(in4)
  Subsystem33/4(out3) -> unpack_status/4(out_pkt_len_err_cnt)
  Subsystem33/3(out2) -> unpack_status/3(out_pad_err_cnt)
  Subsystem33/2(out1) -> unpack_status/2(out_header_err_cnt)
  Subsystem33/1(out0) -> unpack_status/1(out_magic_err_cnt)
  [cnt_rst] -> Subsystem4/1(rst), Subsystem33/1(rst)
  Logical4/1 -> Subsystem4/2(in0)
  Subsystem4/1(out0) -> unpack_status1/1(out_pkt_cnt)
  [upg_sp_dv] -> Logical4/2
  [upg_sp_eof] -> Logical4/1
  Slice17/1 -> local_time_lsw/1(out_timestamp_lsw)
  Slice15/1 -> Convert1/1
  [local_time_capture] -> Delay31/1
  unpack/5(spead_timestamp) -> [spead_timestamp]
  pipeline16/1(q) -> Slice17/1, Slice15/1
  [local_time_src] -> Mux/1
  [time80_48] -> Delay9/1
  [valid80] -> Delay9/2
  [pfb_time] -> Delay10/1
  [pfb_dv] -> Delay10/2
  [flag_dvalid] -> Delay11/2
  [pack_sync_time] -> Delay11/1
  Convert1/1 -> local_time_msw/1(out_timestamp_msw)
  AddSub/1 -> Relational4/2, Relational2/1, time_difference/1(out_time_difference), pipeline204/1(d)
  Logical/1 -> [time_diff_error]
  time_check/1(in_max_difference) -> Relational2/2
  [time_diff_check_en] -> Logical/2
  sync_gen/6(waiting) -> [sync_armed]
  Delay31/1 -> Register3/2, Register2/2, Register4/2, Register1/2
  Delay10/1 -> Register2/1
  [spead_timestamp] -> Register4/1
  Register4/1 -> Mux/2
  Register1/1 -> Mux/3
  Register2/1 -> Mux/4
  Register3/1 -> Mux/5
  Mux/1 -> pipeline16/1(d)
  unpack/4(recvd) -> ts_tvg/6(recvd_in)
  unpack/1(d160) -> ts_tvg/3(data_in)
  unpack/2(dv) -> ts_tvg/4(dv_in)
  unpack/3(time) -> ts_tvg/5(time_in)
  pipeline11/1(q) -> [unpack_d160]
  pipeline12/1(q) -> [unpack_dv]
  pipeline15/1(q) -> [unpack_timestamp]
  ts_tvg/1(d160) -> pipeline11/1(d)
  ts_tvg/2(dv) -> pipeline12/1(d)
  ts_tvg/3(time) -> pipeline15/1(d)
  ts_tvg/4(recvd) -> Terminator9/1
  [ts_tvg_en] -> ts_tvg/1(tvg_en)
  [pipeline_stall] -> ts_tvg/2(stall_pipeline)
  edge_detect4/1(out) -> pipeline5/1(d)
  control/7(in_cnt_rst) -> edge_detect1/1(in)
  edge_detect1/1(out) -> pipeline14/1(d)
  control/3(in_gbe_rst) -> pipeline6/1(d)
  control/1(in_sys_rst) -> pipeline3/1(d)
  pipeline3/1(q) -> [sys_rst]
  pipeline5/1(q) -> [clr_status]
  pipeline6/1(q) -> [gbe_rst]
  pipeline7/1(q) -> [gbe_txen]
  pipeline13/1(q) -> [tvg_adc0_en]
  pipeline14/1(q) -> [cnt_rst]
  control/5(in_tvg_adc0) -> pipeline13/1(d)
  edge_detect2/1(out) -> pipeline38/1(d)
  pipeline38/1(q) -> [gbe_cnt_rst]
  control/8(in_gbe_cnt_rst) -> edge_detect2/1(in)
  control/4(in_gbe_txen) -> pipeline7/1(d)
  control/2(in_status_clr) -> edge_detect4/1(in)
  pipeline43/1(q) -> [adc_snap_arm]
  control/9(in_adc_snap_arm) -> pipeline43/1(d)
  control/10(in_adc_snap_trig_select) -> pipeline39/1(d)
  pipeline39/1(q) -> [adc_snap_trig_source]
  pipeline59/1(q) -> [ct_tvg_en]
  control/11(in_ct_tvg_en) -> pipeline59/1(d)
  pipeline52/1(q) -> [up_dbg_rst]
  control/12(in_unpack_debug_reset) -> pipeline52/1(d)
  control/13(in_cd_bypass) -> pipeline131/1(d)
  pipeline131/1(q) -> [cd_bypass]
  pipeline93/1(q) -> [tvg_adc1_en]
  control/6(in_tvg_adc1) -> pipeline93/1(d)
  control/14(in_gbe_stopmux) -> pipeline9/1(d)
  pipeline9/1(q) -> [gbe_stopmux]
  control/15(in_pfb_bypass) -> pipeline66/1(d)
  pipeline66/1(q) -> [pfb_bypass]
  control/16(in_ts_tvg_en) -> pipeline148/1(d)
  pipeline148/1(q) -> [ts_tvg_en]
  control/17(in_force_gbe_txen) -> pipeline2/1(d)
  pipeline2/1(q) -> [force_gbe_txen]
  control/18(in_snap_stop_mux_sel) -> pipeline127/1(d)
  control/19(in_snap_reord_mux_we_sel) -> pipeline128/1(d)
  pipeline127/1(q) -> [snap_stop_mux_sel]
  pipeline128/1(q) -> [snap_reord_mux_we_sel]
  control/20(in_local_time_source) -> pipeline10/1(d)
  edge_detect6/1(out) -> pipeline164/1(d)
  pipeline164/1(q) -> [local_time_capture]
  pipeline10/1(q) -> [local_time_src]
  control/21(in_local_time_capture) -> edge_detect6/1(in)
  control/22(in_time_diff_check_en) -> pipeline47/1(d)
  pipeline47/1(q) -> [time_diff_check_en]
  control/23(in_auto_rst_enable) -> pipeline132/1(d)
  pipeline132/1(q) -> [auto_rst_enable]
  pipeline155/1(q) -> [pipeline_stall]
  control/24(in_pipeline_stall) -> pipeline155/1(d)
  [board_in_fault] -> Inverter/1
  Inverter/1 -> Logical7/1
  [unpack_timestamp] -> Relational1/1, Delay32/1
  [sys_relock] -> Delay35/1
  [unpack_dv] -> Delay32/2, Delay33/1
  Delay32/1 -> Relational1/2
  Delay35/1 -> snap_sync_gen/13(trig)
  Delay36/1 -> snap_sync_gen/14(stop)
  [sync80] -> Delay36/1
  Logical13/1 -> snap_sync_gen/12(we)
  Delay33/1 -> Logical13/2
  Relational1/1 -> Logical13/1
  [unpack_timestamp] -> Delay46/1
  [cnt_rst] -> Subsystem2/1(rst)
  [synced] -> Delay38/1
  [sync_armed] -> Delay39/1
  [synced] -> Delay45/1
  [sync_armed] -> Delay44/1
  [time_diff_error] -> Delay42/1
  [up_timestep_error] -> Delay41/1
  [cd_error] -> Delay40/1
  [ct_error] -> Delay37/1
  Delay37/1 -> snap_sync_gen/11(in_ct_err)
  Delay40/1 -> snap_sync_gen/10(in_cd_err)
  Delay41/1 -> snap_sync_gen/9(in_timestep_err)
  Delay42/1 -> snap_sync_gen/8(in_time_diff_err)
  Delay44/1 -> snap_sync_gen/7(in_sync_armed)
  Delay45/1 -> snap_sync_gen/6(in_synced)
  Delay46/1 -> snap_sync_gen/5(in_time)
  [up_timestep_error] -> Logical15/1
  [sys_rst] -> Logical9/1
  Logical9/1 -> edge_detect17/1(in)
  [time_diff_error] -> Logical15/4
  [cd_error] -> Logical15/2
  [ct_error] -> Logical15/3
  edge_detect17/1(out) -> [sys_relock], Register/2
  [pack_sync] -> Register/3, Register/1
  Counter3/1 -> Slice13/1
  Slice13/1 -> edge_detect8/1(in)
  Logical15/1 -> [fault_detected]
  Register6/1 -> Inverter2/1
  Register/1 -> posedge_delay1/1(In1), [synced], posedge_delay/1(In1)
  posedge_delay/1(Out1) -> [synced_delay]
  [board_in_fault] -> Delay48/1
  Delay49/1 -> snap_sync_gen/4(in_board_in_fault)
  [board_in_fault] -> Delay49/1
  [synced] -> Inverter1/1
  Inverter1/1 -> Counter1/2
  [pack_sync] -> Counter1/1
  Counter1/1 -> Slice16/1
  Slice16/1 -> edge_detect7/1(in)
  [q_sync] -> Subsystem19/5(in3)
  [pfb_sync] -> Subsystem19/3(in1)
  [fdfs_sync] -> Subsystem19/4(in2)
  [sync80] -> Subsystem19/2(in0)
  [cnt_rst] -> Subsystem19/1(rst)
  Subsystem19/2(out1) -> sync_status2/2(out_sync_pfb_cnt)
  Subsystem19/1(out0) -> sync_status2/1(out_sync80_cnt)
  Subsystem19/3(out2) -> sync_status2/3(out_sync_fdfs_cnt)
  Subsystem19/4(out3) -> sync_status2/4(out_sync_quant_cnt)
  [pack_sync] -> Subsystem9/4(in2)
  [flag_sync] -> Subsystem9/3(in1)
  [ct_sync] -> Subsystem9/2(in0)
  [cnt_rst] -> Subsystem9/1(rst)
  [resync_allow] -> Subsystem2/2(armed)
  [sync_timeout] -> Subsystem2/3(in1)
  [time_diff_error] -> Subsystem2/4(in2)
  [up_timestep_error] -> Subsystem2/5(in3)
  [cd_error] -> Subsystem2/6(in4)
  [ct_error] -> Subsystem2/7(in5)
  Delay48/1 -> sync_status0/2(out_board_in_fault)
  Delay38/1 -> sync_status0/3(out_synced)
  Delay39/1 -> sync_status0/4(out_sync_armed)
  Subsystem9/1(out0) -> sync_status0/5(out_sync_ct)
  Subsystem9/2(out1) -> sync_status0/6(out_sync_flag)
  Subsystem9/3(out2) -> sync_status0/7(out_sync_pack)
  [pack_sync] -> Delay54/1
  [sync_timeout] -> Delay55/1
  Delay54/1 -> snap_sync_gen/3(in_pack_sync)
  Delay55/1 -> snap_sync_gen/2(in_sync_timeout)
  Subsystem2/5(Out5) -> sync_status1/5(out_ct_resync_cnt)
  Subsystem2/1(Out1) -> sync_status1/1(out_timeout_resync_cnt)
  Subsystem2/2(Out2) -> sync_status1/2(out_time_diff_resync_cnt)
  Subsystem2/3(Out3) -> sync_status1/3(out_timestep_resync_cnt)
  Subsystem2/4(Out4) -> sync_status1/4(out_cd_resync_cnt)
  [synced_delay] -> Delay56/1
  Delay56/1 -> snap_sync_gen/1(in_synced_delay)
  [sys_relock] -> Delay57/1
  Inverter2/1 -> [board_in_fault]
  Delay57/1 -> Register6/2
  [synced_delay] -> edge_detect9/1(in)
  edge_detect9/1(out) -> Register6/3, Register6/1
  [synced_delay] -> Delay58/1
  Delay58/1 -> sync_status0/1(out_synced_delay)
  edge_detect7/1(out) -> [sync_timeout]
  [auto_rst_enable] -> Logical8/1
  [resync_allow] -> Logical8/2
  [fault_detected] -> Logical8/3
  [auto_rst_enable] -> Logical14/1
  Logical14/1 -> Logical9/2
  Logical8/1 -> Logical9/3
  [fault_detected] -> Counter5/1
  Counter5/1 -> Slice20/1
  Slice20/1 -> edge_detect10/1(in), Inverter3/1
  Inverter3/1 -> Counter5/2
  [fault_detected] -> Counter3/1
  edge_detect10/1(out) -> [fault_clear_timeout]
  [sync_timeout] -> Logical10/1
  [fault_clear_timeout] -> Logical10/2
  Logical10/1 -> Logical14/2
  edge_detect8/1(out) -> [fault_present_timeout]
  [fault_present_timeout] -> Logical10/3
  posedge_delay1/1(Out1) -> [resync_allow]
  Subsystem2/6(Out6) -> sync_status1/6(out_fault_clear_timeout_cnt)
  Subsystem2/7(Out7) -> sync_status1/7(out_fault_present_timeout_cnt)
  [fault_clear_timeout] -> Subsystem2/8(in6)
  [fault_present_timeout] -> Subsystem2/9(in7)
  Constant3/1 -> Relational4/1
  Relational4/1 -> Logical2/1
  Relational2/1 -> Logical2/2
  Logical2/1 -> Logical/1
  Concat5/1 -> time_gen_cd/6(rd_misc_in)
  time_gen_cd/4(rd_misc_out) -> bus_expand2/1(bus_in)
  [sync_tl_cd0] -> time_gen_cd/1(wr_sync_in)
  [dvalid_tl_cd0] -> time_gen_cd/2(wr_en)
  [hmc_sync_p0] -> time_gen_cd/4(rd_sync_in)
  [hmc_dvalid] -> time_gen_cd/5(rd_en)
  time_gen_cd/1(rd_sync_out) -> [tg_rd_sync]
  time_gen_cd/2(rd_dvalid) -> [tg_rd_dvalid]
  [time80_tl_cd0] -> Slice9/1
  Slice9/1 -> time_gen_cd/3(wr_val_in)
  Constant35/1 -> Concat7/2
  time_gen_cd/3(rd_val_out) -> Concat7/1
  Concat7/1 -> [tg_rd_time_out]
  [hmc_data_p0] -> Concat5/1
  [hmc_data_p1] -> Concat5/2
  bus_expand2/1(msb_out2) -> [tg_data_p0]
  bus_expand2/2(lsb_out1) -> [tg_data_p1]
  [hmc_dvalid] -> Subsystem26/1(In1)
  [dvalid_tl_cd0] -> Subsystem25/1(In1)
  trig_time_msw/1(in_msw) -> pipeline28/1(d)
  trig_time_lsw/1(in_lsw) -> pipeline44/1(d)
  Concat13/1 -> Relational10/1
  pipeline28/1(q) -> Concat13/1
  pipeline44/1(q) -> Concat13/2
  From_pfb_d2/1 -> Relational10/2
  pipeline57/1(q) -> bus_expand7/1(bus_in)
  From142/1 -> pipeline163/1(d)
  From107/1 -> Slice5/1
  Slice14/1 -> pipeline162/1(d)
  From113/1 -> Slice14/1
  pipeline162/1(q) -> snap_adc0/14(extra_timestamp)
  Slice5/1 -> pipeline161/1(d)
  From242/1 -> pipeline57/1(d)
  bus_expand7/4(out5) -> snap_adc0/4(in_p0_d3)
  bus_expand7/5(out4) -> snap_adc0/5(in_p0_d4)
  bus_expand7/1(msb_out8) -> snap_adc0/1(in_p0_d0)
  bus_expand7/2(out7) -> snap_adc0/2(in_p0_d1)
  bus_expand7/3(out6) -> snap_adc0/3(in_p0_d2)
  bus_expand7/6(out3) -> snap_adc0/6(in_p0_d5)
  bus_expand7/7(out2) -> snap_adc0/7(in_p0_d6)
  bus_expand7/8(lsb_out1) -> snap_adc0/8(in_p0_d7)
  pipeline161/1(q) -> snap_adc0/9(in_dv), snap_adc0/11(we)
  Relational10/1 -> Logical12/1
  From243/1 -> pipeline126/1(d)
  Logical12/1 -> snap_adc1/10(trig), snap_adc0/12(trig)
  pipeline163/1(q) -> bus_expand1/1(bus_in)
  bus_expand1/3(out6) -> snap_adc1/3(in_p1_d2)
  bus_expand1/4(out5) -> snap_adc1/4(in_p1_d3)
  bus_expand1/2(out7) -> snap_adc1/2(in_p1_d1)
  bus_expand1/1(msb_out8) -> snap_adc1/1(in_p1_d0)
  bus_expand1/5(out4) -> snap_adc1/5(in_p1_d4)
  bus_expand1/6(out3) -> snap_adc1/6(in_p1_d5)
  bus_expand1/7(out2) -> snap_adc1/7(in_p1_d6)
  bus_expand1/8(lsb_out1) -> snap_adc1/8(in_p1_d7)
  From110/1 -> Slice1/1
  Slice1/1 -> pipeline30/1(d)
  pipeline30/1(q) -> snap_adc1/9(we)
  Slice10/1 -> pipeline32/1(d)
  From327/1 -> Slice10/1
  pipeline32/1(q) -> snap_adc1/12(extra_timestamp)
  pipeline126/1(q) -> Logical12/2
  Delay98/1 -> adc_trig/1(adc_data_p0)
  From240/1 -> Delay98/1
  adc_trig/1(trig) -> Delay105/1
  trig_level/1(in_level) -> Delay100/1
  Delay105/1 -> snap_adc1/11(stop), snap_adc0/13(stop)
  Delay100/1 -> adc_trig/3(trig_pnt)
  From91/1 -> Delay99/1
  Delay99/1 -> adc_trig/2(adc_data_p1)
  [ld_val0] -> pipeline73/1(d)
  [clr_status] -> pipeline25/1(d), pipeline75/1(d)
  tl_cd0/6(time) -> [time80_tl_cd0]
  Constant6/1 -> Concat15/2
  Concat15/1 -> pipeline24/1(d), Gateway Out7/1, pipeline74/1(d)
  [time80] -> Concat15/1
  pipeline75/1(q) -> tl_cd0/1(rst)
  pipeline74/1(q) -> tl_cd0/2(current_time)
  pipeline73/1(q) -> tl_cd0/3(load_value)
  pipeline72/1(q) -> tl_cd0/4(sync_in)
  pipeline71/1(q) -> tl_cd0/5(din)
  pipeline76/1(q) -> tl_cd0/6(en)
  [sync80] -> pipeline36/1(d), pipeline72/1(d)
  [valid80] -> pipeline34/1(d), pipeline76/1(d)
  Constant16/1 -> tl_cd0/7(misci)
  tl_cd0/7(misco) -> Terminator/1
  tl_cd0/3(sync_out) -> [sync_tl_cd0]
  tl_cd0/5(dvalid) -> [dvalid_tl_cd0]
  tl_cd0/4(dout) -> [dout_tl_cd0]
  tl_cd0/2(enable) -> [en_tl_cd0]
  tl_cd0/1(value) -> [delay_tl_cd0]
  pipeline92/1(q) -> tl_cd0/10(load_time)
  pipeline91/1(q) -> tl_cd0/9(load_immediate)
  pipeline90/1(q) -> tl_cd0/8(arm)
  [tl_cd0_arm] -> pipeline90/1(d)
  [tl_cd0_load_immediate] -> pipeline91/1(d)
  [tl_cd0_load_time] -> pipeline92/1(d)
  Gateway Out7/1 -> To Workspace7/1
  [d80_adc0] -> pipeline71/1(d)
  [dvalid_tl_cd0] -> Delay27/1
  [sync_tl_cd0] -> Delay30/1
  [en_tl_cd0] -> Delay25/1
  [delay_tl_cd0] -> Delay26/1
  [dvalid_tl_bs0] -> wb_prog_delay/4(en)
  [delay_tl_bs0] -> wb_prog_delay/2(delay_val)
  [delay_tl_sync0] -> wb_prog_delay/1(sync)
  [en_tl_bs0] -> wb_prog_delay/5(load_val)
  wb_prog_delay/2(data_out) -> [delay_d0]
  wb_prog_delay/3(dvalid) -> [delay_dv]
  wb_prog_delay/1(sync_out) -> [delay_sync]
  pipeline77/1(q) -> tl_cd_bs0/1(rst)
  pipeline1/1(q) -> tl_cd_bs0/2(current_time)
  pipeline78/1(q) -> tl_cd_bs0/3(load_value)
  pipeline84/1(q) -> tl_cd_bs0/4(sync_in)
  pipeline88/1(q) -> tl_cd_bs0/5(din)
  pipeline89/1(q) -> tl_cd_bs0/6(en)
  [clr_status] -> pipeline77/1(d)
  [tg_rd_time_out] -> pipeline1/1(d)
  [ld_val0] -> pipeline78/1(d)
  [tg_rd_sync] -> pipeline84/1(d)
  [tg_rd_dvalid] -> pipeline89/1(d)
  Constant34/1 -> tl_cd_bs0/7(misci)
  tl_cd_bs0/7(misco) -> Terminator12/1
  tl_cd_bs0/4(dout) -> [data_tl_bs0]
  tl_cd_bs0/6(time) -> Terminator13/1
  tl_cd_bs0/5(dvalid) -> [dvalid_tl_bs0]
  tl_cd_bs0/1(value) -> [delay_tl_bs0]
  tl_cd_bs0/3(sync_out) -> [delay_tl_sync0]
  tl_cd_bs0/2(enable) -> [en_tl_bs0]
  pipeline21/1(q) -> tl_cd_bs0/8(arm)
  pipeline22/1(q) -> tl_cd_bs0/9(load_immediate)
  pipeline23/1(q) -> tl_cd_bs0/10(load_time)
  [tl_cd0_arm] -> pipeline21/1(d)
  [tl_cd0_load_immediate] -> pipeline22/1(d)
  [tl_cd0_load_time] -> pipeline23/1(d)
  [data_tl_bs0] -> wb_prog_delay/3(din)
  [tg_data_p0] -> pipeline88/1(d)
  pipeline25/1(q) -> tl_cd1/1(rst)
  [ld_val1] -> pipeline26/1(d)
  pipeline24/1(q) -> tl_cd1/2(current_time)
  pipeline26/1(q) -> tl_cd1/3(load_value)
  pipeline36/1(q) -> tl_cd1/4(sync_in)
  pipeline33/1(q) -> tl_cd1/5(din)
  pipeline34/1(q) -> tl_cd1/6(en)
  pipeline37/1(q) -> tl_cd1/9(load_immediate)
  pipeline35/1(q) -> tl_cd1/8(arm)
  pipeline40/1(q) -> tl_cd1/10(load_time)
  [tl_cd1_arm] -> pipeline35/1(d)
  [tl_cd1_load_immediate] -> pipeline37/1(d)
  [tl_cd1_load_time] -> pipeline40/1(d)
  Constant17/1 -> tl_cd1/7(misci)
  tl_cd1/1(value) -> [delay_tl_cd1]
  tl_cd1/2(enable) -> [en_tl_cd1]
  tl_cd1/3(sync_out) -> [sync_tl_cd1]
  tl_cd1/4(dout) -> [dout_tl_cd1]
  tl_cd1/5(dvalid) -> [dvalid_tl_cd1]
  tl_cd1/6(time) -> [time80_tl_cd1]
  tl_cd1/7(misco) -> Terminator1/1
  [delay_tl_cd1] -> Delay21/1
  [en_tl_cd1] -> Delay28/1
  [sync_tl_cd1] -> Delay24/1
  [dvalid_tl_cd1] -> Delay22/1
  pipeline54/1(q) -> tl_cd_bs1/1(rst)
  pipeline53/1(q) -> tl_cd_bs1/2(current_time)
  pipeline60/1(q) -> tl_cd_bs1/3(load_value)
  pipeline61/1(q) -> tl_cd_bs1/4(sync_in)
  pipeline67/1(q) -> tl_cd_bs1/5(din)
  pipeline68/1(q) -> tl_cd_bs1/6(en)
  [clr_status] -> pipeline54/1(d)
  [tg_rd_time_out] -> pipeline53/1(d)
  [ld_val1] -> pipeline60/1(d)
  [tg_rd_sync] -> pipeline61/1(d)
  [tg_rd_dvalid] -> pipeline68/1(d)
  [tg_data_p1] -> pipeline67/1(d)
  Constant36/1 -> tl_cd_bs1/7(misci)
  pipeline156/1(q) -> tl_cd_bs1/8(arm)
  pipeline69/1(q) -> tl_cd_bs1/9(load_immediate)
  pipeline70/1(q) -> tl_cd_bs1/10(load_time)
  [tl_cd1_load_time] -> pipeline70/1(d)
  [tl_cd1_load_immediate] -> pipeline69/1(d)
  [tl_cd1_arm] -> pipeline156/1(d)
  tl_cd_bs1/7(misco) -> Terminator10/1
  tl_cd_bs1/4(dout) -> [data_tl_bs1]
  tl_cd_bs1/6(time) -> Terminator7/1
  tl_cd_bs1/5(dvalid) -> [dvalid_tl_bs1]
  tl_cd_bs1/1(value) -> [delay_tl_bs1]
  tl_cd_bs1/3(sync_out) -> [delay_tl_sync1]
  tl_cd_bs1/2(enable) -> [en_tl_bs1]
  [delay_tl_sync1] -> wb_prog_delay1/1(sync)
  [delay_tl_bs1] -> wb_prog_delay1/2(delay_val)
  [en_tl_bs1] -> wb_prog_delay1/5(load_val)
  [data_tl_bs1] -> wb_prog_delay1/3(din)
  [dvalid_tl_bs1] -> wb_prog_delay1/4(en)
  wb_prog_delay1/2(data_out) -> [delay_d1]
  wb_prog_delay1/1(sync_out) -> Terminator16/1
  wb_prog_delay1/3(dvalid) -> Terminator11/1
  [d80_adc1] -> pipeline33/1(d)
  Delay30/1 -> cd_hmc/1(sync_in)
  Delay27/1 -> cd_hmc/3(en)
  Delay26/1 -> cd_hmc/4(delay_val)
  Delay25/1 -> cd_hmc/5(load_val)
  [dout_tl_cd0] -> Delay29/1
  Delay29/1 -> cd_hmc/2(din)
  [dout_tl_cd1] -> Delay23/1
  Delay24/1 -> cd_hmc/6(sync_in1)
  Delay23/1 -> cd_hmc/7(din1)
  Delay22/1 -> cd_hmc/8(en1)
  Delay21/1 -> cd_hmc/9(delay_val1)
  Delay28/1 -> cd_hmc/10(load_val1)
  sync_mangle/1(sync_out) -> [hmc_sync_p0]
  sync_mangle/2(dout0) -> [hmc_data_p0]
  sync_mangle/4(dvalid) -> [hmc_dvalid]
  cd_hmc/1(sync_out) -> Delay8/1, sync_mangle/1(sync_in)
  cd_hmc/2(dout0) -> sync_mangle/2(din)
  cd_hmc/4(dvalid) -> sync_mangle/4(en)
  cd_hmc/5(hmc_error) -> [cd_error]
  cd_hmc/3(dout1) -> sync_mangle/3(din1)
  sync_mangle/3(dout1) -> [hmc_data_p1]
  Delay8/1 -> [hmc_sync_raw]
  Delay72/1 -> [flag_sync]
  Delay75/1 -> [flag_misc]
  Delay73/1 -> [flag_dvalid]
  Delay74/1 -> [flag_time]
  Delay43/1 -> time_gen1/4(rd_sync_in)
  Delay59/1 -> time_gen1/6(rd_misc_in)
  Delay/1 -> Delay43/1  "gapsync"
  Delay3/1 -> Delay47/1  "gapdata"
  Mux1/1 -> Delay59/1  "gapvalid"
  [time80] -> Slice2/1
  Delay47/1 -> time_gen1/5(rd_en)
  time_gen1/1(rd_sync_out) -> Delay72/1
  time_gen1/4(rd_misc_out) -> Delay75/1
  time_gen1/2(rd_dvalid) -> Delay73/1
  time_gen1/3(rd_val_out) -> Delay74/1
  [ct_tvg_en2] -> Mux1/1
  Delay17/1 -> Mux1/2
  Delay18/1 -> tvg/1(sync), Delay/1
  Delay16/1 -> tvg/2(dv), Delay3/1
  tvg/1(data256) -> Mux1/3
  [flag_dvalid] -> Subsystem13/1(In1)
  Subsystem13/1(Out1) -> pack_in_dv_rate/1(out_dv_rate)
  [s256_v] -> Subsystem11/1(In1)
  Subsystem11/1(Out1) -> pack_out_dv_rate/1(out_dv_rate)
  pipeline121/1(q) -> Convert/1
  pipeline124/1(q) -> [ip_per_x]
  pipeline125/1(q) -> [num_x]
  x_setup/1(in_f_per_x) -> pipeline121/1(d)
  x_setup/2(in_ip_per_x) -> pipeline124/1(d)
  x_setup/3(in_num_x) -> pipeline125/1(d)
  pipeline120/1(q) -> [pack_snap_arm]
  x_setup/4(in_snap_arm) -> pipeline120/1(d)
  pipeline130/1(q) -> [pktstart_sel]
  x_setup/5(in_pktstart_mux) -> pipeline130/1(d)
  [s256_v] -> pack_block_check/1(dv)
  [cnt_rst] -> Subsystem14/1(rst)
  Subsystem14/1(out0) -> pack_dv_err/1(out_dvblock_err_cnt)
  pack_block_check/1(error) -> [pack_dv_err], Subsystem14/2(in0)
  pipeline149/1(q) -> [pack_mux]
  x_setup/6(in_pack_mux) -> pipeline149/1(d)
  Convert/1 -> [f_per_x]
  [ct_d256] -> Delay17/1
  [ct_dv] -> Delay16/1
  [ct_sync] -> Delay18/1
  x_setup/7(in_pktoffset_sel) -> pipeline63/1(d)
  pipeline63/1(q) -> [pktoffset_sel]
  iptx_base/1(in_reg) -> pipeline105/1(d)
  pipeline105/1(q) -> [tx_ip_base]
  tx_metadata/1(in_porttx) -> pipeline106/1(d)
  tx_metadata/2(in_board_id) -> pipeline107/1(d)
  pipeline106/1(q) -> [tx_port]
  pipeline107/1(q) -> [tx_board_id]
  pipeline17/1(q) -> [outfreq_stopmux]
  ct_debug/6(in_outfreq_stopmux) -> pipeline17/1(d)
  pipeline18/1(q) -> [out_stopmux]
  ct_debug/5(in_out_stopmux) -> pipeline18/1(d)
  pipeline55/1(q) -> [wrrd_stopmux]
  ct_debug/3(in_wrrd_stopmux) -> pipeline55/1(d)
  pipeline56/1(q) -> [in_stopmux]
  ct_debug/1(in_in_stopmux) -> pipeline56/1(d)
  pipeline122/1(q) -> [ct_snap_arm]
  pipeline147/1(q) -> edge_detect5/1
  ct_debug/8(in_snap_trig) -> pipeline147/1(d)
  ct_debug/7(in_snap_arm) -> pipeline122/1(d)
  edge_detect5/1 -> [ct_snap_trig]
  ct_debug/2(in_in_trigmux) -> pipeline150/1(d)
  pipeline150/1(q) -> [in_trigmux]
  ct_debug/4(in_obuf_stopmux) -> pipeline167/1(d)
  pipeline167/1(q) -> [obuf_stopmux]
  ct_debug/9(in_snap_wesel) -> pipeline8/1(d)
  pipeline8/1(q) -> [ct_snap_wesel]
  pipeline157/1(q) -> [ct_snap_trigsel]
  ct_debug/10(in_snap_trigsel) -> pipeline157/1(d)
  pipeline166/1(q) -> [ct_snap_circsel]
  ct_debug/11(in_snap_circsel) -> pipeline166/1(d)
  [ct_dv] -> Subsystem8/1(In1)
  [ct_pktstart] -> we_delay1/1(d)
  [ct_dv] -> we_delay2/1(d)
  we_delay1/1(q) -> pktlen_check/1(pkt_start)
  we_delay2/1(q) -> dv_block_check/1(dv), pktlen_check/2(dv)
  pktlen_check/1(error) -> we_delay7/1(d)
  dv_block_check/1(error) -> we_delay29/1(d)
  [cnt_rst] -> Subsystem6/1(rst)
  we_delay7/1(q) -> [ct_pktlen_err], Subsystem6/2(in0)
  we_delay29/1(q) -> [ct_dvblk_err], Subsystem6/3(in1)
  Delay64/1 -> Delay68/1
  Delay4/1 -> Delay5/1
  Delay5/1 -> Delay60/1
  Delay60/1 -> Delay64/1
  Delay68/1 -> [flag_pktstart]
  Delay14/1 -> Delay6/1
  Delay6/1 -> Delay61/1
  Delay65/1 -> Delay69/1
  Delay69/1 -> [flag_pktfreq]
  Delay61/1 -> Delay65/1
  Delay15/1 -> Delay7/1
  Delay7/1 -> Delay62/1
  Delay62/1 -> Delay66/1
  Delay66/1 -> Delay70/1
  Delay70/1 -> [flag_pktxindex]
  Delay19/1 -> Delay20/1
  Delay20/1 -> Delay63/1
  Delay63/1 -> Delay67/1
  Delay67/1 -> Delay71/1
  Delay71/1 -> [flag_pktxoffset]
  [ct_pkt_x_index] -> Delay15/1
  [ct_pkt_x_offset] -> Delay19/1
  [ct_pktfreq] -> Delay14/1
  [ct_pktstart] -> Delay4/1
  [flag_sync] -> packetiser/1(sync_in)
  [flag_dvalid] -> packetiser/2(en)
  [flag_pktstart] -> packetiser/5(pkt_start)
  [flag_pktxoffset] -> packetiser/7(pkt_x_offset)
  [tx_ip_base] -> packetiser/9(base_ip)
  [tx_port] -> packetiser/10(base_port)
  Constant28/1 -> concat1/2
  [flag_time] -> concat1/1
  [flag_misc] -> packetiser/3(din)
  concat1/1 -> [pack_sync_time], packetiser/4(timestamp)
  Delay82/1 -> [s256_d]
  Delay83/1 -> [s256_v]
  Delay84/1 -> [s256_eof]
  Delay85/1 -> [s256_of]
  Delay86/1 -> [s256_ip]
  Delay87/1 -> [s256_port]
  Delay88/1 -> [pack_sync]
  packetiser/1(dout) -> Delay82/1
  packetiser/2(dvalid) -> Delay83/1
  packetiser/3(eof) -> Delay84/1
  packetiser/4(overflow) -> Delay85/1
  packetiser/5(destination_ip) -> Delay86/1
  packetiser/6(destination_port) -> Delay87/1
  packetiser/7(sync) -> Delay88/1
  [flag_pktfreq] -> Delay77/1
  Delay89/1 -> [s256_pktfreq]
  Delay77/1 -> Delay89/1
  [flag_pktxindex] -> Delay78/1
  Delay78/1 -> Delay90/1
  Delay90/1 -> [s256_pktxindex]
  [flag_pktxoffset] -> Delay79/1
  Delay79/1 -> Delay91/1
  Delay91/1 -> [s256_pktxoffset]
  [tx_board_id] -> packetiser/8(board_id)
  [flag_pktstart] -> Delay80/1
  Delay80/1 -> Delay92/1
  Delay92/1 -> [s256_pktstart]
  [sync80] -> time_gen1/1(wr_sync_in)
  [valid80] -> time_gen1/2(wr_en)
  [sync80] -> Subsystem/2(sync)
  [valid80] -> Subsystem/3(dv)
  Subsystem/1(msw) -> sync_time_msw/1(out_reg)
  Subsystem/2(ls32) -> sync_time_lsw/1(out_reg)
  [q_dv] -> Subsystem17/1(In1)
  [flag_pktxindex] -> packetiser/6(pkt_x_index)
  [flag_time] -> Delay81/1
  Delay81/1 -> Delay93/1
  Delay93/1 -> [s256_time]
  time_gen1/5(epoch) -> Delay76/1
  Slice4/1 -> flag_epoch_lsw/1(out_reg)
  Slice11/1 -> flag_epoch_msw/1(out_reg)
  Delay76/1 -> Concat10/1
  Constant8/1 -> Concat10/2
  Concat10/1 -> Slice4/1, Slice11/1, [flag_epoch]
  [q_sync] -> hmc_ct/1(in_sync)
  [q_dv] -> hmc_ct/2(in_dv)
  [q_d64_0] -> hmc_ct/3(in_d0)
  [q_d64_1] -> hmc_ct/4(in_d1)
  hmc_ct/1(out_sync) -> [ct_sync]
  hmc_ct/2(out_dv) -> [ct_dv]
  hmc_ct/3(out_d256) -> [ct_d256]
  hmc_ct/4(pkt_start) -> [ct_pktstart]
  hmc_ct/5(freq_id) -> [ct_pktfreq]
  hmc_ct/6(x_index) -> [ct_pkt_x_index]
  hmc_ct/7(x_pkt_index) -> [ct_pkt_x_offset]
  hmc_ct/8(error0) -> [ct_error]
  [cnt_rst] -> Subsystem10/1(rst)
  [q_sync] -> Subsystem10/2(in0)
  Constant/1 -> Subsystem10/3(in1)
  Constant9/1 -> Subsystem10/4(in2)
